simulink model "solar_pv_protected_c07_circuit"  (R2026b)
(part 4 of 16)

      | 用語9　　　　　　　 ; GND：Ground（回路の基準電位・電流帰路）。この図の共通基準。保護接地や大地への接続を意味するとは限らない。
      | 用語10　　　　　　　; AGND：Analog Ground（アナログ回路の基準端子）。アナログ部分の電流帰路。現図では共通GNDへ接続されるが、実装時の電流経路への配慮は別途必要。
      | 用語11　　　　　　　; DGND：Digital Ground（デジタル回路の基準端子）。デジタル部分の電流帰路。現図では共通GNDへ接続される。
      | 用語12　　　　　　　; VREF/REF：基準電圧を表す端子名。REFはReference（基準）の意味。ADCの変換尺度や電流アンプの出力基準に使う。REF1/REF2の接続電位は個別に確認する。
      | 用語13　　　　　　　; VCC/VDD/VEE/VS：ICの電源端子名。文字の歴史的な由来を現在の接続機能へ当てはめない。現回路のVEEはU8/U10では浮動基準SW、U9ではGND。各電圧・基準は端子と接続を参照する。
      | 用語14　　　　　　　; GNDP：U10の一次側電源の基準端子。絶縁電源の入力側GND。二次側基準VEE=SWと直接同一の導体ではない。
      | 用語15　　　　　　　; SW：Switching Node（スイッチング点）。主電力段の上下MOSFETとL1がつながる、電圧が高速に切り替わる点。GNDとは別電位。
  GND_Label_043 : ConnectionLabel  Description=|  Label=GND
      | この回路での名前　　; GND
      | 種別　　　　　　　　; ConnectionLabel
      | この回路での役割　　; 電池BT1の負極、太陽電池列の負極、制御・測定・保護回路のGNDを結ぶ共通の帰路。高側駆動の浮動帰路SWとは別のノード。
      | 共通帰路の代表接続　; BT1（充電先の蓄電池／51.2V 100Ah LiFePO4）: -
      |                     ; PV1（直列太陽電池列の負極側パネル／400W panel 1/2）: -
      |                     ; U7（RP2040搭載Pico W／SC0918）: 3(GND), 8(GND), 13(GND), 18(GND), 23(GND), 28(GND), 33(AGND), 38(GND)
      |                     ; U1（外付けADC／MCP3208-CI/SL）: 8(CH7), 9(DGND), 14(AGND)
      |                     ; P_U1（保護MOSFETを制御する保護IC／LTC4364IMS-1#PBF）: GND
      |                     ; Q2（同期整流降圧回路の下側スイッチ／TK9R6E15Q5,S1X）: 3(S)
      |                     ; U9（低側の光ゲートドライバ／ACPL-P346-560E）: 4(VEE)
      |                     ; U10（高側ゲート用の浮動電源を作る絶縁DC/DC／UCC14131QDWNRQ1）: 1(GNDP), 2(GNDP), 5(GNDP), 8(GNDP), 9(GNDP), 10(GNDP), 11(GNDP), 12(GNDP), 13(GNDP), 14(GNDP), 15(GNDP), 16(GNDP), 17(GNDP), 18(GNDP)
      | この場所の直接接続　; C7（入力フィルム／3.3 uF）: 2(n)
      | 直接接続の範囲　　　; このラベルから実際の線・分岐・明示的な境界端子だけを追った接続。同名ラベルによる離れた場所への接続はこの欄に含めない。
      | 同一ネット全端子　　; BT1: -
      |                     ; C1: 2(n)
      |                     ; C2: 2(n)
      |                     ; C3: 2(n)
      |                     ; C4: 2(n)
      |                     ; C7: 2(n)
      |                     ; C8: 2(n)
      |                     ; C9: 2(n)
      |                     ; C10: 2(n)
      |                     ; C13: 2(n)
      |                     ; C14: 2(n)
      |                     ; C15: 2(n)
      |                     ; C16: 2(n)
      |                     ; C17: 2
      |                     ; C18: 2
      |                     ; C19: 2
      |                     ; C20: 2
      |                     ; C21: 2
      |                     ; C22: 2
      |                     ; C23: 2
      |                     ; C24: 2
      |                     ; C25: 2
      |                     ; C26: 2
      |                     ; C27: 2
      |                     ; C28: 2
      |                     ; C29: 2
      |                     ; C30: 2
      |                     ; C31: 2
      |                     ; C33: 2
      |                     ; C34: 2
      |                     ; C35: 2
      |                     ; C36: 2
      |                     ; C40: 2
      |                     ; C41: 2
      |                     ; C42: 2
      |                     ; C43: 2
      |                     ; C44: 2
      |                     ; C45: 2
      |                     ; C46: 2
      |                     ; C47: 2
      |                     ; C48: 2
      |                     ; D2: 2(A)
      |                     ; PV1: -
      |                     ; P_CHG: N
      |                     ; P_COUT: N
      |                     ; P_CTMR: N
      |                     ; P_D1: A
      |                     ; P_R3: 2
      |                     ; P_R8: 2
      |                     ; P_RSHDN_PD: 2
      |                     ; P_U1: GND
      |                     ; Q2: 3(S)
      |                     ; Q3: 1(S1), 4(S2)
      |                     ; R1: 2(n)
      |                     ; R18: 2
      |                     ; R21: 2
      |                     ; R24: 2
      |                     ; R35: 2
      |                     ; R42: 2
      |                     ; R44: 2
      |                     ; R48: 2
      |                     ; U1: 8(CH7), 9(DGND), 14(AGND)
      |                     ; U2: 2(GND), 3(REF2), 4(RESERVED_GND)
      |                     ; U3: 2(GND), 3(REF2), 4(RESERVED_GND)
      |                     ; U4: 3(GND)
      |                     ; U5: 3(GND)
      |                     ; U6: 3(GND)
      |                     ; U7: 3(GND), 8(GND), 13(GND), 18(GND), 23(GND), 28(GND), 33(AGND), 38(GND)
      |                     ; U9: 4(VEE)
      |                     ; U10: 1(GNDP), 2(GNDP), 5(GNDP), 8(GNDP), 9(GNDP), 10(GNDP), 11(GNDP), 12(GNDP), 13(GNDP), 14(GNDP), 15(GNDP), 16(GNDP), 17(GNDP), 18(GNDP)
      |                     ; U11: 2(GND)
      |                     ; U12: 2(GND)
      | 接続部品数　　　　　; 72部品（部品番号で集計。同一ネット全体）
      | 接続端子数　　　　　; 99端子（423端子の部品対応表で集計。ラベル・境界ポートの重複は含めない）
      | この場所の端子数　　; 1端子／1部品（同名ラベルによる接続を除く）
      | 同階層同名ラベル数　; 75個（このラベル自身を含む）
      | 全階層の接続ラベル　; 87個（実際に同じノードへつながるラベル。名前が違う別名も含む）
      | 接続ルール　　　　　; 同じ階層の同じラベル名を仮想配線として結ぶ。別のSubsystem内とは名前だけでつながらず、明示的なConnection Portと配線をたどる。色は用途の表示であり接続を決めない。
      | 確認の範囲　　　　　; 現在の保存回路の端子・配線から求めた静的接続。抵抗やICの内部を導線として短絡せずに集計した。説明の更新は動作シミュレーション、タイミング、実部品の性能・実機動作を保証するものではない。
      | 記録の基準　　　　　; measurement_label_layout_20261022_r01/after_layout_graph.json。部品対応表は端子名の対応付けにのみ使用。
      | 
      | 【この説明欄の略語・記号】
      | 用語1　　　　　　　 ; DC：Direct Current（直流）。ここでは直流電源または直流成分。DCバイアスはコンデンサに重なる直流電圧を指す。
      | 用語2　　　　　　　 ; DC/DC：DC-to-DC Converter（直流電圧変換器）。直流入力を別の直流電圧へ変換する電源回路。絶縁の有無は個々の部品説明で確認する。
      | 用語3　　　　　　　 ; ADC：Analog-to-Digital Converter（アナログ・デジタル変換器）。測定電圧をデジタル値へ変換する回路。電流や温度も、センサーで電圧へ変換した後に読み取る。
      | 用語4　　　　　　　 ; IC：Integrated Circuit（集積回路）。複数の電子素子と機能を小さな半導体チップに集積した部品。
      | 用語5　　　　　　　 ; CH：Channel（測定チャネル）。CH0〜CH7はADCの入力番号であり、同時測定を意味しない。
      | 用語6　　　　　　　 ; MOSFET：Metal-Oxide-Semiconductor Field-Effect Transistor（金属・酸化膜・半導体構造の電界効果トランジスタ）。ゲートとソースの電圧でドレインとソースの導通を制御する素子。N-MOSはNチャネル型を表す。
      | 用語7　　　　　　　 ; LiFePO4：Lithium Iron Phosphate（リン酸鉄リチウム）。電池の正極材料を示す化学式。英語の頭文字を並べた略語ではない。
      | 用語8　　　　　　　 ; GND：Ground（回路の基準電位・電流帰路）。この図の共通基準。保護接地や大地への接続を意味するとは限らない。
      | 用語9　　　　　　　 ; AGND：Analog Ground（アナログ回路の基準端子）。アナログ部分の電流帰路。現図では共通GNDへ接続されるが、実装時の電流経路への配慮は別途必要。
      | 用語10　　　　　　　; DGND：Digital Ground（デジタル回路の基準端子）。デジタル部分の電流帰路。現図では共通GNDへ接続される。
      | 用語11　　　　　　　; VREF/REF：基準電圧を表す端子名。REFはReference（基準）の意味。ADCの変換尺度や電流アンプの出力基準に使う。REF1/REF2の接続電位は個別に確認する。
      | 用語12　　　　　　　; VCC/VDD/VEE/VS：ICの電源端子名。文字の歴史的な由来を現在の接続機能へ当てはめない。現回路のVEEはU8/U10では浮動基準SW、U9ではGND。各電圧・基準は端子と接続を参照する。
      | 用語13　　　　　　　; GNDP：U10の一次側電源の基準端子。絶縁電源の入力側GND。二次側基準VEE=SWと直接同一の導体ではない。
      | 用語14　　　　　　　; SW：Switching Node（スイッチング点）。主電力段の上下MOSFETとL1がつながる、電圧が高速に切り替わる点。GNDとは別電位。
  GND_Label_044 : ConnectionLabel  Description=|  Label=GND
      | この回路での名前　　; GND
      | 種別　　　　　　　　; ConnectionLabel
      | この回路での役割　　; 電池BT1の負極、太陽電池列の負極、制御・測定・保護回路のGNDを結ぶ共通の帰路。高側駆動の浮動帰路SWとは別のノード。
      | 共通帰路の代表接続　; BT1（充電先の蓄電池／51.2V 100Ah LiFePO4）: -
      |                     ; PV1（直列太陽電池列の負極側パネル／400W panel 1/2）: -
      |                     ; U7（RP2040搭載Pico W／SC0918）: 3(GND), 8(GND), 13(GND), 18(GND), 23(GND), 28(GND), 33(AGND), 38(GND)
      |                     ; U1（外付けADC／MCP3208-CI/SL）: 8(CH7), 9(DGND), 14(AGND)
      |                     ; P_U1（保護MOSFETを制御する保護IC／LTC4364IMS-1#PBF）: GND
      |                     ; Q2（同期整流降圧回路の下側スイッチ／TK9R6E15Q5,S1X）: 3(S)
      |                     ; U9（低側の光ゲートドライバ／ACPL-P346-560E）: 4(VEE)
      |                     ; U10（高側ゲート用の浮動電源を作る絶縁DC/DC／UCC14131QDWNRQ1）: 1(GNDP), 2(GNDP), 5(GNDP), 8(GNDP), 9(GNDP), 10(GNDP), 11(GNDP), 12(GNDP), 13(GNDP), 14(GNDP), 15(GNDP), 16(GNDP), 17(GNDP), 18(GNDP)
      | この場所の直接接続　; C8（入力高速バイパス／2.2 uF）: 2(n)
      | 直接接続の範囲　　　; このラベルから実際の線・分岐・明示的な境界端子だけを追った接続。同名ラベルによる離れた場所への接続はこの欄に含めない。
      | 同一ネット全端子　　; BT1: -
      |                     ; C1: 2(n)
      |                     ; C2: 2(n)
      |                     ; C3: 2(n)
      |                     ; C4: 2(n)
      |                     ; C7: 2(n)
      |                     ; C8: 2(n)
      |                     ; C9: 2(n)
      |                     ; C10: 2(n)
      |                     ; C13: 2(n)
      |                     ; C14: 2(n)
      |                     ; C15: 2(n)
      |                     ; C16: 2(n)
      |                     ; C17: 2
      |                     ; C18: 2
      |                     ; C19: 2
      |                     ; C20: 2
      |                     ; C21: 2
      |                     ; C22: 2
      |                     ; C23: 2
      |                     ; C24: 2
      |                     ; C25: 2
      |                     ; C26: 2
      |                     ; C27: 2
      |                     ; C28: 2
      |                     ; C29: 2
      |                     ; C30: 2
      |                     ; C31: 2
      |                     ; C33: 2
      |                     ; C34: 2
      |                     ; C35: 2
      |                     ; C36: 2
      |                     ; C40: 2
      |                     ; C41: 2
      |                     ; C42: 2
      |                     ; C43: 2
      |                     ; C44: 2
      |                     ; C45: 2
      |                     ; C46: 2
      |                     ; C47: 2
      |                     ; C48: 2
      |                     ; D2: 2(A)
      |                     ; PV1: -
      |                     ; P_CHG: N
      |                     ; P_COUT: N
      |                     ; P_CTMR: N
      |                     ; P_D1: A
      |                     ; P_R3: 2
      |                     ; P_R8: 2
      |                     ; P_RSHDN_PD: 2
      |                     ; P_U1: GND
      |                     ; Q2: 3(S)
      |                     ; Q3: 1(S1), 4(S2)
      |                     ; R1: 2(n)
      |                     ; R18: 2
      |                     ; R21: 2
      |                     ; R24: 2
      |                     ; R35: 2
      |                     ; R42: 2
      |                     ; R44: 2
      |                     ; R48: 2
      |                     ; U1: 8(CH7), 9(DGND), 14(AGND)
      |                     ; U2: 2(GND), 3(REF2), 4(RESERVED_GND)
      |                     ; U3: 2(GND), 3(REF2), 4(RESERVED_GND)
      |                     ; U4: 3(GND)
      |                     ; U5: 3(GND)
      |                     ; U6: 3(GND)
      |                     ; U7: 3(GND), 8(GND), 13(GND), 18(GND), 23(GND), 28(GND), 33(AGND), 38(GND)
      |                     ; U9: 4(VEE)
      |                     ; U10: 1(GNDP), 2(GNDP), 5(GNDP), 8(GNDP), 9(GNDP), 10(GNDP), 11(GNDP), 12(GNDP), 13(GNDP), 14(GNDP), 15(GNDP), 16(GNDP), 17(GNDP), 18(GNDP)
      |                     ; U11: 2(GND)
      |                     ; U12: 2(GND)
      | 接続部品数　　　　　; 72部品（部品番号で集計。同一ネット全体）
      | 接続端子数　　　　　; 99端子（423端子の部品対応表で集計。ラベル・境界ポートの重複は含めない）
      | この場所の端子数　　; 1端子／1部品（同名ラベルによる接続を除く）
      | 同階層同名ラベル数　; 75個（このラベル自身を含む）
      | 全階層の接続ラベル　; 87個（実際に同じノードへつながるラベル。名前が違う別名も含む）
      | 接続ルール　　　　　; 同じ階層の同じラベル名を仮想配線として結ぶ。別のSubsystem内とは名前だけでつながらず、明示的なConnection Portと配線をたどる。色は用途の表示であり接続を決めない。
      | 確認の範囲　　　　　; 現在の保存回路の端子・配線から求めた静的接続。抵抗やICの内部を導線として短絡せずに集計した。説明の更新は動作シミュレーション、タイミング、実部品の性能・実機動作を保証するものではない。
      | 記録の基準　　　　　; measurement_label_layout_20261022_r01/after_layout_graph.json。部品対応表は端子名の対応付けにのみ使用。
      | 
      | 【この説明欄の略語・記号】
      | 用語1　　　　　　　 ; DC：Direct Current（直流）。ここでは直流電源または直流成分。DCバイアスはコンデンサに重なる直流電圧を指す。
      | 用語2　　　　　　　 ; DC/DC：DC-to-DC Converter（直流電圧変換器）。直流入力を別の直流電圧へ変換する電源回路。絶縁の有無は個々の部品説明で確認する。
      | 用語3　　　　　　　 ; ADC：Analog-to-Digital Converter（アナログ・デジタル変換器）。測定電圧をデジタル値へ変換する回路。電流や温度も、センサーで電圧へ変換した後に読み取る。
      | 用語4　　　　　　　 ; IC：Integrated Circuit（集積回路）。複数の電子素子と機能を小さな半導体チップに集積した部品。
      | 用語5　　　　　　　 ; CH：Channel（測定チャネル）。CH0〜CH7はADCの入力番号であり、同時測定を意味しない。
      | 用語6　　　　　　　 ; MOSFET：Metal-Oxide-Semiconductor Field-Effect Transistor（金属・酸化膜・半導体構造の電界効果トランジスタ）。ゲートとソースの電圧でドレインとソースの導通を制御する素子。N-MOSはNチャネル型を表す。
      | 用語7　　　　　　　 ; LiFePO4：Lithium Iron Phosphate（リン酸鉄リチウム）。電池の正極材料を示す化学式。英語の頭文字を並べた略語ではない。
      | 用語8　　　　　　　 ; GND：Ground（回路の基準電位・電流帰路）。この図の共通基準。保護接地や大地への接続を意味するとは限らない。
      | 用語9　　　　　　　 ; AGND：Analog Ground（アナログ回路の基準端子）。アナログ部分の電流帰路。現図では共通GNDへ接続されるが、実装時の電流経路への配慮は別途必要。
      | 用語10　　　　　　　; DGND：Digital Ground（デジタル回路の基準端子）。デジタル部分の電流帰路。現図では共通GNDへ接続される。
      | 用語11　　　　　　　; VREF/REF：基準電圧を表す端子名。REFはReference（基準）の意味。ADCの変換尺度や電流アンプの出力基準に使う。REF1/REF2の接続電位は個別に確認する。
      | 用語12　　　　　　　; VCC/VDD/VEE/VS：ICの電源端子名。文字の歴史的な由来を現在の接続機能へ当てはめない。現回路のVEEはU8/U10では浮動基準SW、U9ではGND。各電圧・基準は端子と接続を参照する。
      | 用語13　　　　　　　; GNDP：U10の一次側電源の基準端子。絶縁電源の入力側GND。二次側基準VEE=SWと直接同一の導体ではない。
      | 用語14　　　　　　　; SW：Switching Node（スイッチング点）。主電力段の上下MOSFETとL1がつながる、電圧が高速に切り替わる点。GNDとは別電位。
  GND_Label_045 : ConnectionLabel  Description=|  Label=GND
      | この回路での名前　　; GND
      | 種別　　　　　　　　; ConnectionLabel
      | この回路での役割　　; 電池BT1の負極、太陽電池列の負極、制御・測定・保護回路のGNDを結ぶ共通の帰路。高側駆動の浮動帰路SWとは別のノード。
      | 共通帰路の代表接続　; BT1（充電先の蓄電池／51.2V 100Ah LiFePO4）: -
      |                     ; PV1（直列太陽電池列の負極側パネル／400W panel 1/2）: -
      |                     ; U7（RP2040搭載Pico W／SC0918）: 3(GND), 8(GND), 13(GND), 18(GND), 23(GND), 28(GND), 33(AGND), 38(GND)
      |                     ; U1（外付けADC／MCP3208-CI/SL）: 8(CH7), 9(DGND), 14(AGND)
      |                     ; P_U1（保護MOSFETを制御する保護IC／LTC4364IMS-1#PBF）: GND
      |                     ; Q2（同期整流降圧回路の下側スイッチ／TK9R6E15Q5,S1X）: 3(S)
      |                     ; U9（低側の光ゲートドライバ／ACPL-P346-560E）: 4(VEE)
      |                     ; U10（高側ゲート用の浮動電源を作る絶縁DC/DC／UCC14131QDWNRQ1）: 1(GNDP), 2(GNDP), 5(GNDP), 8(GNDP), 9(GNDP), 10(GNDP), 11(GNDP), 12(GNDP), 13(GNDP), 14(GNDP), 15(GNDP), 16(GNDP), 17(GNDP), 18(GNDP)
      | この場所の直接接続　; C9（入力高速バイパス／2.2 uF）: 2(n)
      | 直接接続の範囲　　　; このラベルから実際の線・分岐・明示的な境界端子だけを追った接続。同名ラベルによる離れた場所への接続はこの欄に含めない。
      | 同一ネット全端子　　; BT1: -
      |                     ; C1: 2(n)
      |                     ; C2: 2(n)
      |                     ; C3: 2(n)
      |                     ; C4: 2(n)
      |                     ; C7: 2(n)
      |                     ; C8: 2(n)
      |                     ; C9: 2(n)
      |                     ; C10: 2(n)
      |                     ; C13: 2(n)
      |                     ; C14: 2(n)
      |                     ; C15: 2(n)
      |                     ; C16: 2(n)
      |                     ; C17: 2
      |                     ; C18: 2
      |                     ; C19: 2
      |                     ; C20: 2
      |                     ; C21: 2
      |                     ; C22: 2
      |                     ; C23: 2
      |                     ; C24: 2
      |                     ; C25: 2
      |                     ; C26: 2
      |                     ; C27: 2
      |                     ; C28: 2
      |                     ; C29: 2
      |                     ; C30: 2
      |                     ; C31: 2
      |                     ; C33: 2
      |                     ; C34: 2
      |                     ; C35: 2
      |                     ; C36: 2
      |                     ; C40: 2
      |                     ; C41: 2
      |                     ; C42: 2
      |                     ; C43: 2
      |                     ; C44: 2
      |                     ; C45: 2
      |                     ; C46: 2
      |                     ; C47: 2
      |                     ; C48: 2
      |                     ; D2: 2(A)
      |                     ; PV1: -
      |                     ; P_CHG: N
      |                     ; P_COUT: N
      |                     ; P_CTMR: N
      |                     ; P_D1: A
      |                     ; P_R3: 2
      |                     ; P_R8: 2
      |                     ; P_RSHDN_PD: 2
      |                     ; P_U1: GND
      |                     ; Q2: 3(S)
      |                     ; Q3: 1(S1), 4(S2)
      |                     ; R1: 2(n)
      |                     ; R18: 2
      |                     ; R21: 2
      |                     ; R24: 2
      |                     ; R35: 2
      |                     ; R42: 2
      |                     ; R44: 2
      |                     ; R48: 2
      |                     ; U1: 8(CH7), 9(DGND), 14(AGND)
      |                     ; U2: 2(GND), 3(REF2), 4(RESERVED_GND)
      |                     ; U3: 2(GND), 3(REF2), 4(RESERVED_GND)
      |                     ; U4: 3(GND)
      |                     ; U5: 3(GND)
      |                     ; U6: 3(GND)
      |                     ; U7: 3(GND), 8(GND), 13(GND), 18(GND), 23(GND), 28(GND), 33(AGND), 38(GND)
      |                     ; U9: 4(VEE)
      |                     ; U10: 1(GNDP), 2(GNDP), 5(GNDP), 8(GNDP), 9(GNDP), 10(GNDP), 11(GNDP), 12(GNDP), 13(GNDP), 14(GNDP), 15(GNDP), 16(GNDP), 17(GNDP), 18(GNDP)
      |                     ; U11: 2(GND)
      |                     ; U12: 2(GND)
      | 接続部品数　　　　　; 72部品（部品番号で集計。同一ネット全体）
      | 接続端子数　　　　　; 99端子（423端子の部品対応表で集計。ラベル・境界ポートの重複は含めない）
      | この場所の端子数　　; 1端子／1部品（同名ラベルによる接続を除く）
      | 同階層同名ラベル数　; 75個（このラベル自身を含む）
      | 全階層の接続ラベル　; 87個（実際に同じノードへつながるラベル。名前が違う別名も含む）
      | 接続ルール　　　　　; 同じ階層の同じラベル名を仮想配線として結ぶ。別のSubsystem内とは名前だけでつながらず、明示的なConnection Portと配線をたどる。色は用途の表示であり接続を決めない。
      | 確認の範囲　　　　　; 現在の保存回路の端子・配線から求めた静的接続。抵抗やICの内部を導線として短絡せずに集計した。説明の更新は動作シミュレーション、タイミング、実部品の性能・実機動作を保証するものではない。
      | 記録の基準　　　　　; measurement_label_layout_20261022_r01/after_layout_graph.json。部品対応表は端子名の対応付けにのみ使用。
      | 
      | 【この説明欄の略語・記号】
      | 用語1　　　　　　　 ; DC：Direct Current（直流）。ここでは直流電源または直流成分。DCバイアスはコンデンサに重なる直流電圧を指す。
      | 用語2　　　　　　　 ; DC/DC：DC-to-DC Converter（直流電圧変換器）。直流入力を別の直流電圧へ変換する電源回路。絶縁の有無は個々の部品説明で確認する。
      | 用語3　　　　　　　 ; ADC：Analog-to-Digital Converter（アナログ・デジタル変換器）。測定電圧をデジタル値へ変換する回路。電流や温度も、センサーで電圧へ変換した後に読み取る。
      | 用語4　　　　　　　 ; IC：Integrated Circuit（集積回路）。複数の電子素子と機能を小さな半導体チップに集積した部品。
      | 用語5　　　　　　　 ; CH：Channel（測定チャネル）。CH0〜CH7はADCの入力番号であり、同時測定を意味しない。
      | 用語6　　　　　　　 ; MOSFET：Metal-Oxide-Semiconductor Field-Effect Transistor（金属・酸化膜・半導体構造の電界効果トランジスタ）。ゲートとソースの電圧でドレインとソースの導通を制御する素子。N-MOSはNチャネル型を表す。
      | 用語7　　　　　　　 ; LiFePO4：Lithium Iron Phosphate（リン酸鉄リチウム）。電池の正極材料を示す化学式。英語の頭文字を並べた略語ではない。
      | 用語8　　　　　　　 ; GND：Ground（回路の基準電位・電流帰路）。この図の共通基準。保護接地や大地への接続を意味するとは限らない。
      | 用語9　　　　　　　 ; AGND：Analog Ground（アナログ回路の基準端子）。アナログ部分の電流帰路。現図では共通GNDへ接続されるが、実装時の電流経路への配慮は別途必要。
      | 用語10　　　　　　　; DGND：Digital Ground（デジタル回路の基準端子）。デジタル部分の電流帰路。現図では共通GNDへ接続される。
      | 用語11　　　　　　　; VREF/REF：基準電圧を表す端子名。REFはReference（基準）の意味。ADCの変換尺度や電流アンプの出力基準に使う。REF1/REF2の接続電位は個別に確認する。
      | 用語12　　　　　　　; VCC/VDD/VEE/VS：ICの電源端子名。文字の歴史的な由来を現在の接続機能へ当てはめない。現回路のVEEはU8/U10では浮動基準SW、U9ではGND。各電圧・基準は端子と接続を参照する。
      | 用語13　　　　　　　; GNDP：U10の一次側電源の基準端子。絶縁電源の入力側GND。二次側基準VEE=SWと直接同一の導体ではない。
      | 用語14　　　　　　　; SW：Switching Node（スイッチング点）。主電力段の上下MOSFETとL1がつながる、電圧が高速に切り替わる点。GNDとは別電位。
  GND_Label_046 : ConnectionLabel  Description=|  Label=GND
      | この回路での名前　　; GND
      | 種別　　　　　　　　; ConnectionLabel
      | この回路での役割　　; 電池BT1の負極、太陽電池列の負極、制御・測定・保護回路のGNDを結ぶ共通の帰路。高側駆動の浮動帰路SWとは別のノード。
      | 共通帰路の代表接続　; BT1（充電先の蓄電池／51.2V 100Ah LiFePO4）: -
      |                     ; PV1（直列太陽電池列の負極側パネル／400W panel 1/2）: -
      |                     ; U7（RP2040搭載Pico W／SC0918）: 3(GND), 8(GND), 13(GND), 18(GND), 23(GND), 28(GND), 33(AGND), 38(GND)
      |                     ; U1（外付けADC／MCP3208-CI/SL）: 8(CH7), 9(DGND), 14(AGND)
      |                     ; P_U1（保護MOSFETを制御する保護IC／LTC4364IMS-1#PBF）: GND
      |                     ; Q2（同期整流降圧回路の下側スイッチ／TK9R6E15Q5,S1X）: 3(S)
      |                     ; U9（低側の光ゲートドライバ／ACPL-P346-560E）: 4(VEE)
      |                     ; U10（高側ゲート用の浮動電源を作る絶縁DC/DC／UCC14131QDWNRQ1）: 1(GNDP), 2(GNDP), 5(GNDP), 8(GNDP), 9(GNDP), 10(GNDP), 11(GNDP), 12(GNDP), 13(GNDP), 14(GNDP), 15(GNDP), 16(GNDP), 17(GNDP), 18(GNDP)
      | この場所の直接接続　; D2（Q2のゲート–ソース間電圧が過大になるのを抑えるため、GATE_L–GND間へ配置する／15V gate clamp）: 2(A)
      |                     ; Q2（同期整流降圧回路の下側スイッチ／TK9R6E15Q5,S1X）: 3(S)
      |                     ; R44（Q2のゲートをソースGNDへ戻し、ドライバ未給電時の残留電荷を逃がす／10k 1%）: 2
      | 直接接続の範囲　　　; このラベルから実際の線・分岐・明示的な境界端子だけを追った接続。同名ラベルによる離れた場所への接続はこの欄に含めない。
      | 同一ネット全端子　　; BT1: -
      |                     ; C1: 2(n)
      |                     ; C2: 2(n)
      |                     ; C3: 2(n)
      |                     ; C4: 2(n)
      |                     ; C7: 2(n)
      |                     ; C8: 2(n)
      |                     ; C9: 2(n)
      |                     ; C10: 2(n)
      |                     ; C13: 2(n)
      |                     ; C14: 2(n)
      |                     ; C15: 2(n)
      |                     ; C16: 2(n)
      |                     ; C17: 2
      |                     ; C18: 2
      |                     ; C19: 2
      |                     ; C20: 2
      |                     ; C21: 2
      |                     ; C22: 2
      |                     ; C23: 2
      |                     ; C24: 2
      |                     ; C25: 2
      |                     ; C26: 2
      |                     ; C27: 2
      |                     ; C28: 2
      |                     ; C29: 2
      |                     ; C30: 2
      |                     ; C31: 2
      |                     ; C33: 2
      |                     ; C34: 2
      |                     ; C35: 2
      |                     ; C36: 2
      |                     ; C40: 2
      |                     ; C41: 2
      |                     ; C42: 2
      |                     ; C43: 2
      |                     ; C44: 2
      |                     ; C45: 2
      |                     ; C46: 2
      |                     ; C47: 2
      |                     ; C48: 2
      |                     ; D2: 2(A)
      |                     ; PV1: -
      |                     ; P_CHG: N
      |                     ; P_COUT: N
      |                     ; P_CTMR: N
      |                     ; P_D1: A
      |                     ; P_R3: 2
      |                     ; P_R8: 2
      |                     ; P_RSHDN_PD: 2
      |                     ; P_U1: GND
      |                     ; Q2: 3(S)
      |                     ; Q3: 1(S1), 4(S2)
      |                     ; R1: 2(n)
      |                     ; R18: 2
      |                     ; R21: 2
      |                     ; R24: 2
      |                     ; R35: 2
      |                     ; R42: 2
      |                     ; R44: 2
      |                     ; R48: 2
      |                     ; U1: 8(CH7), 9(DGND), 14(AGND)
      |                     ; U2: 2(GND), 3(REF2), 4(RESERVED_GND)
      |                     ; U3: 2(GND), 3(REF2), 4(RESERVED_GND)
      |                     ; U4: 3(GND)
      |                     ; U5: 3(GND)
      |                     ; U6: 3(GND)
      |                     ; U7: 3(GND), 8(GND), 13(GND), 18(GND), 23(GND), 28(GND), 33(AGND), 38(GND)
      |                     ; U9: 4(VEE)
      |                     ; U10: 1(GNDP), 2(GNDP), 5(GNDP), 8(GNDP), 9(GNDP), 10(GNDP), 11(GNDP), 12(GNDP), 13(GNDP), 14(GNDP), 15(GNDP), 16(GNDP), 17(GNDP), 18(GNDP)
      |                     ; U11: 2(GND)
      |                     ; U12: 2(GND)
      | 接続部品数　　　　　; 72部品（部品番号で集計。同一ネット全体）
      | 接続端子数　　　　　; 99端子（423端子の部品対応表で集計。ラベル・境界ポートの重複は含めない）
      | この場所の端子数　　; 3端子／3部品（同名ラベルによる接続を除く）
      | 同階層同名ラベル数　; 75個（このラベル自身を含む）
      | 全階層の接続ラベル　; 87個（実際に同じノードへつながるラベル。名前が違う別名も含む）
      | 接続ルール　　　　　; 同じ階層の同じラベル名を仮想配線として結ぶ。別のSubsystem内とは名前だけでつながらず、明示的なConnection Portと配線をたどる。色は用途の表示であり接続を決めない。
      | 確認の範囲　　　　　; 現在の保存回路の端子・配線から求めた静的接続。抵抗やICの内部を導線として短絡せずに集計した。説明の更新は動作シミュレーション、タイミング、実部品の性能・実機動作を保証するものではない。
      | 記録の基準　　　　　; measurement_label_layout_20261022_r01/after_layout_graph.json。部品対応表は端子名の対応付けにのみ使用。
      | 
      | 【この説明欄の略語・記号】
      | 用語1　　　　　　　 ; DC：Direct Current（直流）。ここでは直流電源または直流成分。DCバイアスはコンデンサに重なる直流電圧を指す。
      | 用語2　　　　　　　 ; DC/DC：DC-to-DC Converter（直流電圧変換器）。直流入力を別の直流電圧へ変換する電源回路。絶縁の有無は個々の部品説明で確認する。
      | 用語3　　　　　　　 ; ADC：Analog-to-Digital Converter（アナログ・デジタル変換器）。測定電圧をデジタル値へ変換する回路。電流や温度も、センサーで電圧へ変換した後に読み取る。
      | 用語4　　　　　　　 ; IC：Integrated Circuit（集積回路）。複数の電子素子と機能を小さな半導体チップに集積した部品。
      | 用語5　　　　　　　 ; CH：Channel（測定チャネル）。CH0〜CH7はADCの入力番号であり、同時測定を意味しない。
      | 用語6　　　　　　　 ; MOSFET：Metal-Oxide-Semiconductor Field-Effect Transistor（金属・酸化膜・半導体構造の電界効果トランジスタ）。ゲートとソースの電圧でドレインとソースの導通を制御する素子。N-MOSはNチャネル型を表す。
      | 用語7　　　　　　　 ; LiFePO4：Lithium Iron Phosphate（リン酸鉄リチウム）。電池の正極材料を示す化学式。英語の頭文字を並べた略語ではない。
      | 用語8　　　　　　　 ; GND：Ground（回路の基準電位・電流帰路）。この図の共通基準。保護接地や大地への接続を意味するとは限らない。
      | 用語9　　　　　　　 ; AGND：Analog Ground（アナログ回路の基準端子）。アナログ部分の電流帰路。現図では共通GNDへ接続されるが、実装時の電流経路への配慮は別途必要。
      | 用語10　　　　　　　; DGND：Digital Ground（デジタル回路の基準端子）。デジタル部分の電流帰路。現図では共通GNDへ接続される。
      | 用語11　　　　　　　; VREF/REF：基準電圧を表す端子名。REFはReference（基準）の意味。ADCの変換尺度や電流アンプの出力基準に使う。REF1/REF2の接続電位は個別に確認する。
      | 用語12　　　　　　　; VCC/VDD/VEE/VS：ICの電源端子名。文字の歴史的な由来を現在の接続機能へ当てはめない。現回路のVEEはU8/U10では浮動基準SW、U9ではGND。各電圧・基準は端子と接続を参照する。
      | 用語13　　　　　　　; GNDP：U10の一次側電源の基準端子。絶縁電源の入力側GND。二次側基準VEE=SWと直接同一の導体ではない。
      | 用語14　　　　　　　; SW：Switching Node（スイッチング点）。主電力段の上下MOSFETとL1がつながる、電圧が高速に切り替わる点。GNDとは別電位。
  GND_Label_047 : ConnectionLabel  Description=|  Label=GND
      | この回路での名前　　; GND
      | 種別　　　　　　　　; ConnectionLabel
      | この回路での役割　　; 電池BT1の負極、太陽電池列の負極、制御・測定・保護回路のGNDを結ぶ共通の帰路。高側駆動の浮動帰路SWとは別のノード。
      | 共通帰路の代表接続　; BT1（充電先の蓄電池／51.2V 100Ah LiFePO4）: -
      |                     ; PV1（直列太陽電池列の負極側パネル／400W panel 1/2）: -
      |                     ; U7（RP2040搭載Pico W／SC0918）: 3(GND), 8(GND), 13(GND), 18(GND), 23(GND), 28(GND), 33(AGND), 38(GND)
      |                     ; U1（外付けADC／MCP3208-CI/SL）: 8(CH7), 9(DGND), 14(AGND)
      |                     ; P_U1（保護MOSFETを制御する保護IC／LTC4364IMS-1#PBF）: GND
      |                     ; Q2（同期整流降圧回路の下側スイッチ／TK9R6E15Q5,S1X）: 3(S)
      |                     ; U9（低側の光ゲートドライバ／ACPL-P346-560E）: 4(VEE)
      |                     ; U10（高側ゲート用の浮動電源を作る絶縁DC/DC／UCC14131QDWNRQ1）: 1(GNDP), 2(GNDP), 5(GNDP), 8(GNDP), 9(GNDP), 10(GNDP), 11(GNDP), 12(GNDP), 13(GNDP), 14(GNDP), 15(GNDP), 16(GNDP), 17(GNDP), 18(GNDP)
      | この場所の直接接続　; PV1（直列太陽電池列の負極側パネル／400W panel 1/2）: -
      | 直接接続の範囲　　　; このラベルから実際の線・分岐・明示的な境界端子だけを追った接続。同名ラベルによる離れた場所への接続はこの欄に含めない。
      | 同一ネット全端子　　; BT1: -
      |                     ; C1: 2(n)
      |                     ; C2: 2(n)
      |                     ; C3: 2(n)
      |                     ; C4: 2(n)
      |                     ; C7: 2(n)
      |                     ; C8: 2(n)
      |                     ; C9: 2(n)
      |                     ; C10: 2(n)
      |                     ; C13: 2(n)
      |                     ; C14: 2(n)
      |                     ; C15: 2(n)
      |                     ; C16: 2(n)
      |                     ; C17: 2
      |                     ; C18: 2
      |                     ; C19: 2
      |                     ; C20: 2
      |                     ; C21: 2
      |                     ; C22: 2
      |                     ; C23: 2
      |                     ; C24: 2
      |                     ; C25: 2
      |                     ; C26: 2
      |                     ; C27: 2
      |                     ; C28: 2
      |                     ; C29: 2
      |                     ; C30: 2
      |                     ; C31: 2
      |                     ; C33: 2
      |                     ; C34: 2
      |                     ; C35: 2
      |                     ; C36: 2
      |                     ; C40: 2
      |                     ; C41: 2
      |                     ; C42: 2
      |                     ; C43: 2
      |                     ; C44: 2
      |                     ; C45: 2
      |                     ; C46: 2
      |                     ; C47: 2
      |                     ; C48: 2
      |                     ; D2: 2(A)
      |                     ; PV1: -
      |                     ; P_CHG: N
      |                     ; P_COUT: N
      |                     ; P_CTMR: N
      |                     ; P_D1: A
      |                     ; P_R3: 2
      |                     ; P_R8: 2
      |                     ; P_RSHDN_PD: 2
      |                     ; P_U1: GND
      |                     ; Q2: 3(S)
      |                     ; Q3: 1(S1), 4(S2)
      |                     ; R1: 2(n)
      |                     ; R18: 2
      |                     ; R21: 2
      |                     ; R24: 2
      |                     ; R35: 2
      |                     ; R42: 2
      |                     ; R44: 2
      |                     ; R48: 2
      |                     ; U1: 8(CH7), 9(DGND), 14(AGND)
      |                     ; U2: 2(GND), 3(REF2), 4(RESERVED_GND)
      |                     ; U3: 2(GND), 3(REF2), 4(RESERVED_GND)
      |                     ; U4: 3(GND)
      |                     ; U5: 3(GND)
      |                     ; U6: 3(GND)
      |                     ; U7: 3(GND), 8(GND), 13(GND), 18(GND), 23(GND), 28(GND), 33(AGND), 38(GND)
      |                     ; U9: 4(VEE)
      |                     ; U10: 1(GNDP), 2(GNDP), 5(GNDP), 8(GNDP), 9(GNDP), 10(GNDP), 11(GNDP), 12(GNDP), 13(GNDP), 14(GNDP), 15(GNDP), 16(GNDP), 17(GNDP), 18(GNDP)
      |                     ; U11: 2(GND)
      |                     ; U12: 2(GND)
      | 接続部品数　　　　　; 72部品（部品番号で集計。同一ネット全体）
      | 接続端子数　　　　　; 99端子（423端子の部品対応表で集計。ラベル・境界ポートの重複は含めない）
      | この場所の端子数　　; 1端子／1部品（同名ラベルによる接続を除く）
      | 同階層同名ラベル数　; 75個（このラベル自身を含む）
      | 全階層の接続ラベル　; 87個（実際に同じノードへつながるラベル。名前が違う別名も含む）
      | 接続ルール　　　　　; 同じ階層の同じラベル名を仮想配線として結ぶ。別のSubsystem内とは名前だけでつながらず、明示的なConnection Portと配線をたどる。色は用途の表示であり接続を決めない。
      | 確認の範囲　　　　　; 現在の保存回路の端子・配線から求めた静的接続。抵抗やICの内部を導線として短絡せずに集計した。説明の更新は動作シミュレーション、タイミング、実部品の性能・実機動作を保証するものではない。
      | 記録の基準　　　　　; measurement_label_layout_20261022_r01/after_layout_graph.json。部品対応表は端子名の対応付けにのみ使用。
      | 
      | 【この説明欄の略語・記号】
      | 用語1　　　　　　　 ; DC：Direct Current（直流）。ここでは直流電源または直流成分。DCバイアスはコンデンサに重なる直流電圧を指す。
      | 用語2　　　　　　　 ; DC/DC：DC-to-DC Converter（直流電圧変換器）。直流入力を別の直流電圧へ変換する電源回路。絶縁の有無は個々の部品説明で確認する。
      | 用語3　　　　　　　 ; ADC：Analog-to-Digital Converter（アナログ・デジタル変換器）。測定電圧をデジタル値へ変換する回路。電流や温度も、センサーで電圧へ変換した後に読み取る。
      | 用語4　　　　　　　 ; IC：Integrated Circuit（集積回路）。複数の電子素子と機能を小さな半導体チップに集積した部品。
      | 用語5　　　　　　　 ; CH：Channel（測定チャネル）。CH0〜CH7はADCの入力番号であり、同時測定を意味しない。
      | 用語6　　　　　　　 ; MOSFET：Metal-Oxide-Semiconductor Field-Effect Transistor（金属・酸化膜・半導体構造の電界効果トランジスタ）。ゲートとソースの電圧でドレインとソースの導通を制御する素子。N-MOSはNチャネル型を表す。
      | 用語7　　　　　　　 ; LiFePO4：Lithium Iron Phosphate（リン酸鉄リチウム）。電池の正極材料を示す化学式。英語の頭文字を並べた略語ではない。
      | 用語8　　　　　　　 ; GND：Ground（回路の基準電位・電流帰路）。この図の共通基準。保護接地や大地への接続を意味するとは限らない。
      | 用語9　　　　　　　 ; AGND：Analog Ground（アナログ回路の基準端子）。アナログ部分の電流帰路。現図では共通GNDへ接続されるが、実装時の電流経路への配慮は別途必要。
      | 用語10　　　　　　　; DGND：Digital Ground（デジタル回路の基準端子）。デジタル部分の電流帰路。現図では共通GNDへ接続される。
      | 用語11　　　　　　　; VREF/REF：基準電圧を表す端子名。REFはReference（基準）の意味。ADCの変換尺度や電流アンプの出力基準に使う。REF1/REF2の接続電位は個別に確認する。
      | 用語12　　　　　　　; VCC/VDD/VEE/VS：ICの電源端子名。文字の歴史的な由来を現在の接続機能へ当てはめない。現回路のVEEはU8/U10では浮動基準SW、U9ではGND。各電圧・基準は端子と接続を参照する。
      | 用語13　　　　　　　; GNDP：U10の一次側電源の基準端子。絶縁電源の入力側GND。二次側基準VEE=SWと直接同一の導体ではない。
      | 用語14　　　　　　　; SW：Switching Node（スイッチング点）。主電力段の上下MOSFETとL1がつながる、電圧が高速に切り替わる点。GNDとは別電位。
  GND_Label_049 : ConnectionLabel  Description=|  Label=GND
      | この回路での名前　　; GND
      | 種別　　　　　　　　; ConnectionLabel
      | この回路での役割　　; 電池BT1の負極、太陽電池列の負極、制御・測定・保護回路のGNDを結ぶ共通の帰路。高側駆動の浮動帰路SWとは別のノード。
      | 共通帰路の代表接続　; BT1（充電先の蓄電池／51.2V 100Ah LiFePO4）: -
      |                     ; PV1（直列太陽電池列の負極側パネル／400W panel 1/2）: -
      |                     ; U7（RP2040搭載Pico W／SC0918）: 3(GND), 8(GND), 13(GND), 18(GND), 23(GND), 28(GND), 33(AGND), 38(GND)
      |                     ; U1（外付けADC／MCP3208-CI/SL）: 8(CH7), 9(DGND), 14(AGND)
      |                     ; P_U1（保護MOSFETを制御する保護IC／LTC4364IMS-1#PBF）: GND
      |                     ; Q2（同期整流降圧回路の下側スイッチ／TK9R6E15Q5,S1X）: 3(S)
      |                     ; U9（低側の光ゲートドライバ／ACPL-P346-560E）: 4(VEE)
      |                     ; U10（高側ゲート用の浮動電源を作る絶縁DC/DC／UCC14131QDWNRQ1）: 1(GNDP), 2(GNDP), 5(GNDP), 8(GNDP), 9(GNDP), 10(GNDP), 11(GNDP), 12(GNDP), 13(GNDP), 14(GNDP), 15(GNDP), 16(GNDP), 17(GNDP), 18(GNDP)
      | この場所の直接接続　; Q3（RP2040のPWM_Lを受け、U9の入力LED電流をGNDへ引き込む／dual 30V logic-level LED sink）: 1(S1)
      | 直接接続の範囲　　　; このラベルから実際の線・分岐・明示的な境界端子だけを追った接続。同名ラベルによる離れた場所への接続はこの欄に含めない。
      | 同一ネット全端子　　; BT1: -
      |                     ; C1: 2(n)
      |                     ; C2: 2(n)
      |                     ; C3: 2(n)
      |                     ; C4: 2(n)
      |                     ; C7: 2(n)
      |                     ; C8: 2(n)
      |                     ; C9: 2(n)
      |                     ; C10: 2(n)
      |                     ; C13: 2(n)
      |                     ; C14: 2(n)
      |                     ; C15: 2(n)
      |                     ; C16: 2(n)
      |                     ; C17: 2
      |                     ; C18: 2
      |                     ; C19: 2
      |                     ; C20: 2
      |                     ; C21: 2
      |                     ; C22: 2
      |                     ; C23: 2
      |                     ; C24: 2
      |                     ; C25: 2
      |                     ; C26: 2
      |                     ; C27: 2
      |                     ; C28: 2
      |                     ; C29: 2
      |                     ; C30: 2
      |                     ; C31: 2
      |                     ; C33: 2
      |                     ; C34: 2
      |                     ; C35: 2
      |                     ; C36: 2
      |                     ; C40: 2
      |                     ; C41: 2
      |                     ; C42: 2
      |                     ; C43: 2
      |                     ; C44: 2
      |                     ; C45: 2
      |                     ; C46: 2
      |                     ; C47: 2
      |                     ; C48: 2
      |                     ; D2: 2(A)
      |                     ; PV1: -
      |                     ; P_CHG: N
      |                     ; P_COUT: N
      |                     ; P_CTMR: N
      |                     ; P_D1: A
      |                     ; P_R3: 2
      |                     ; P_R8: 2
      |                     ; P_RSHDN_PD: 2
      |                     ; P_U1: GND
      |                     ; Q2: 3(S)
      |                     ; Q3: 1(S1), 4(S2)
      |                     ; R1: 2(n)
      |                     ; R18: 2
      |                     ; R21: 2
      |                     ; R24: 2
      |                     ; R35: 2
      |                     ; R42: 2
      |                     ; R44: 2
      |                     ; R48: 2
      |                     ; U1: 8(CH7), 9(DGND), 14(AGND)
      |                     ; U2: 2(GND), 3(REF2), 4(RESERVED_GND)
      |                     ; U3: 2(GND), 3(REF2), 4(RESERVED_GND)
      |                     ; U4: 3(GND)
      |                     ; U5: 3(GND)
      |                     ; U6: 3(GND)
      |                     ; U7: 3(GND), 8(GND), 13(GND), 18(GND), 23(GND), 28(GND), 33(AGND), 38(GND)
      |                     ; U9: 4(VEE)
      |                     ; U10: 1(GNDP), 2(GNDP), 5(GNDP), 8(GNDP), 9(GNDP), 10(GNDP), 11(GNDP), 12(GNDP), 13(GNDP), 14(GNDP), 15(GNDP), 16(GNDP), 17(GNDP), 18(GNDP)
      |                     ; U11: 2(GND)
      |                     ; U12: 2(GND)
      | 接続部品数　　　　　; 72部品（部品番号で集計。同一ネット全体）
      | 接続端子数　　　　　; 99端子（423端子の部品対応表で集計。ラベル・境界ポートの重複は含めない）
      | この場所の端子数　　; 1端子／1部品（同名ラベルによる接続を除く）
      | 同階層同名ラベル数　; 75個（このラベル自身を含む）
      | 全階層の接続ラベル　; 87個（実際に同じノードへつながるラベル。名前が違う別名も含む）
      | 接続ルール　　　　　; 同じ階層の同じラベル名を仮想配線として結ぶ。別のSubsystem内とは名前だけでつながらず、明示的なConnection Portと配線をたどる。色は用途の表示であり接続を決めない。
      | 確認の範囲　　　　　; 現在の保存回路の端子・配線から求めた静的接続。抵抗やICの内部を導線として短絡せずに集計した。説明の更新は動作シミュレーション、タイミング、実部品の性能・実機動作を保証するものではない。
      | 記録の基準　　　　　; measurement_label_layout_20261022_r01/after_layout_graph.json。部品対応表は端子名の対応付けにのみ使用。
      | 
      | 【この説明欄の略語・記号】
      | 用語1　　　　　　　 ; DC：Direct Current（直流）。ここでは直流電源または直流成分。DCバイアスはコンデンサに重なる直流電圧を指す。
      | 用語2　　　　　　　 ; DC/DC：DC-to-DC Converter（直流電圧変換器）。直流入力を別の直流電圧へ変換する電源回路。絶縁の有無は個々の部品説明で確認する。
      | 用語3　　　　　　　 ; ADC：Analog-to-Digital Converter（アナログ・デジタル変換器）。測定電圧をデジタル値へ変換する回路。電流や温度も、センサーで電圧へ変換した後に読み取る。
      | 用語4　　　　　　　 ; IC：Integrated Circuit（集積回路）。複数の電子素子と機能を小さな半導体チップに集積した部品。
      | 用語5　　　　　　　 ; PWM：Pulse Width Modulation（パルス幅変調）。周期に対するON時間の割合を変えて、スイッチの平均的な電力伝達を調整する方式。
      | 用語6　　　　　　　 ; CH：Channel（測定チャネル）。CH0〜CH7はADCの入力番号であり、同時測定を意味しない。
      | 用語7　　　　　　　 ; MOSFET：Metal-Oxide-Semiconductor Field-Effect Transistor（金属・酸化膜・半導体構造の電界効果トランジスタ）。ゲートとソースの電圧でドレインとソースの導通を制御する素子。N-MOSはNチャネル型を表す。
      | 用語8　　　　　　　 ; LED：Light-Emitting Diode（発光ダイオード）。本回路のゲートドライバ入力では光によって信号を伝え、入力側と出力側を絶縁するために用いる。
      | 用語9　　　　　　　 ; LiFePO4：Lithium Iron Phosphate（リン酸鉄リチウム）。電池の正極材料を示す化学式。英語の頭文字を並べた略語ではない。
      | 用語10　　　　　　　; GND：Ground（回路の基準電位・電流帰路）。この図の共通基準。保護接地や大地への接続を意味するとは限らない。
      | 用語11　　　　　　　; AGND：Analog Ground（アナログ回路の基準端子）。アナログ部分の電流帰路。現図では共通GNDへ接続されるが、実装時の電流経路への配慮は別途必要。
      | 用語12　　　　　　　; DGND：Digital Ground（デジタル回路の基準端子）。デジタル部分の電流帰路。現図では共通GNDへ接続される。
      | 用語13　　　　　　　; VREF/REF：基準電圧を表す端子名。REFはReference（基準）の意味。ADCの変換尺度や電流アンプの出力基準に使う。REF1/REF2の接続電位は個別に確認する。
      | 用語14　　　　　　　; VCC/VDD/VEE/VS：ICの電源端子名。文字の歴史的な由来を現在の接続機能へ当てはめない。現回路のVEEはU8/U10では浮動基準SW、U9ではGND。各電圧・基準は端子と接続を参照する。
      | 用語15　　　　　　　; GNDP：U10の一次側電源の基準端子。絶縁電源の入力側GND。二次側基準VEE=SWと直接同一の導体ではない。
      | 用語16　　　　　　　; SW：Switching Node（スイッチング点）。主電力段の上下MOSFETとL1がつながる、電圧が高速に切り替わる点。GNDとは別電位。
  GND_Label_050 : ConnectionLabel  Description=|  Label=GND
      | この回路での名前　　; GND
      | 種別　　　　　　　　; ConnectionLabel
      | この回路での役割　　; 電池BT1の負極、太陽電池列の負極、制御・測定・保護回路のGNDを結ぶ共通の帰路。高側駆動の浮動帰路SWとは別のノード。
      | 共通帰路の代表接続　; BT1（充電先の蓄電池／51.2V 100Ah LiFePO4）: -
      |                     ; PV1（直列太陽電池列の負極側パネル／400W panel 1/2）: -
      |                     ; U7（RP2040搭載Pico W／SC0918）: 3(GND), 8(GND), 13(GND), 18(GND), 23(GND), 28(GND), 33(AGND), 38(GND)
      |                     ; U1（外付けADC／MCP3208-CI/SL）: 8(CH7), 9(DGND), 14(AGND)
      |                     ; P_U1（保護MOSFETを制御する保護IC／LTC4364IMS-1#PBF）: GND
      |                     ; Q2（同期整流降圧回路の下側スイッチ／TK9R6E15Q5,S1X）: 3(S)
      |                     ; U9（低側の光ゲートドライバ／ACPL-P346-560E）: 4(VEE)
      |                     ; U10（高側ゲート用の浮動電源を作る絶縁DC/DC／UCC14131QDWNRQ1）: 1(GNDP), 2(GNDP), 5(GNDP), 8(GNDP), 9(GNDP), 10(GNDP), 11(GNDP), 12(GNDP), 13(GNDP), 14(GNDP), 15(GNDP), 16(GNDP), 17(GNDP), 18(GNDP)
      | この場所の直接接続　; Q3（RP2040のPWM_Lを受け、U9の入力LED電流をGNDへ引き込む／dual 30V logic-level LED sink）: 4(S2)
      | 直接接続の範囲　　　; このラベルから実際の線・分岐・明示的な境界端子だけを追った接続。同名ラベルによる離れた場所への接続はこの欄に含めない。
      | 同一ネット全端子　　; BT1: -
      |                     ; C1: 2(n)
      |                     ; C2: 2(n)
      |                     ; C3: 2(n)
      |                     ; C4: 2(n)
      |                     ; C7: 2(n)
      |                     ; C8: 2(n)
      |                     ; C9: 2(n)
      |                     ; C10: 2(n)
      |                     ; C13: 2(n)
      |                     ; C14: 2(n)
      |                     ; C15: 2(n)
      |                     ; C16: 2(n)
      |                     ; C17: 2
      |                     ; C18: 2
      |                     ; C19: 2
      |                     ; C20: 2
      |                     ; C21: 2
      |                     ; C22: 2
      |                     ; C23: 2
      |                     ; C24: 2
      |                     ; C25: 2
      |                     ; C26: 2
      |                     ; C27: 2
      |                     ; C28: 2
      |                     ; C29: 2
      |                     ; C30: 2
      |                     ; C31: 2
      |                     ; C33: 2
      |                     ; C34: 2
      |                     ; C35: 2
      |                     ; C36: 2
      |                     ; C40: 2
      |                     ; C41: 2
      |                     ; C42: 2
      |                     ; C43: 2
      |                     ; C44: 2
      |                     ; C45: 2
      |                     ; C46: 2
      |                     ; C47: 2
      |                     ; C48: 2
      |                     ; D2: 2(A)
      |                     ; PV1: -
      |                     ; P_CHG: N
      |                     ; P_COUT: N
      |                     ; P_CTMR: N
      |                     ; P_D1: A
      |                     ; P_R3: 2
      |                     ; P_R8: 2
      |                     ; P_RSHDN_PD: 2
      |                     ; P_U1: GND
      |                     ; Q2: 3(S)
      |                     ; Q3: 1(S1), 4(S2)
      |                     ; R1: 2(n)
      |                     ; R18: 2
      |                     ; R21: 2
      |                     ; R24: 2
      |                     ; R35: 2
      |                     ; R42: 2
      |                     ; R44: 2
      |                     ; R48: 2
      |                     ; U1: 8(CH7), 9(DGND), 14(AGND)
      |                     ; U2: 2(GND), 3(REF2), 4(RESERVED_GND)
      |                     ; U3: 2(GND), 3(REF2), 4(RESERVED_GND)
      |                     ; U4: 3(GND)
      |                     ; U5: 3(GND)
      |                     ; U6: 3(GND)
      |                     ; U7: 3(GND), 8(GND), 13(GND), 18(GND), 23(GND), 28(GND), 33(AGND), 38(GND)
      |                     ; U9: 4(VEE)
      |                     ; U10: 1(GNDP), 2(GNDP), 5(GNDP), 8(GNDP), 9(GNDP), 10(GNDP), 11(GNDP), 12(GNDP), 13(GNDP), 14(GNDP), 15(GNDP), 16(GNDP), 17(GNDP), 18(GNDP)
      |                     ; U11: 2(GND)
      |                     ; U12: 2(GND)
      | 接続部品数　　　　　; 72部品（部品番号で集計。同一ネット全体）
      | 接続端子数　　　　　; 99端子（423端子の部品対応表で集計。ラベル・境界ポートの重複は含めない）
      | この場所の端子数　　; 1端子／1部品（同名ラベルによる接続を除く）
      | 同階層同名ラベル数　; 75個（このラベル自身を含む）
      | 全階層の接続ラベル　; 87個（実際に同じノードへつながるラベル。名前が違う別名も含む）
      | 接続ルール　　　　　; 同じ階層の同じラベル名を仮想配線として結ぶ。別のSubsystem内とは名前だけでつながらず、明示的なConnection Portと配線をたどる。色は用途の表示であり接続を決めない。
      | 確認の範囲　　　　　; 現在の保存回路の端子・配線から求めた静的接続。抵抗やICの内部を導線として短絡せずに集計した。説明の更新は動作シミュレーション、タイミング、実部品の性能・実機動作を保証するものではない。
      | 記録の基準　　　　　; measurement_label_layout_20261022_r01/after_layout_graph.json。部品対応表は端子名の対応付けにのみ使用。
      | 
      | 【この説明欄の略語・記号】
      | 用語1　　　　　　　 ; DC：Direct Current（直流）。ここでは直流電源または直流成分。DCバイアスはコンデンサに重なる直流電圧を指す。
      | 用語2　　　　　　　 ; DC/DC：DC-to-DC Converter（直流電圧変換器）。直流入力を別の直流電圧へ変換する電源回路。絶縁の有無は個々の部品説明で確認する。
      | 用語3　　　　　　　 ; ADC：Analog-to-Digital Converter（アナログ・デジタル変換器）。測定電圧をデジタル値へ変換する回路。電流や温度も、センサーで電圧へ変換した後に読み取る。
      | 用語4　　　　　　　 ; IC：Integrated Circuit（集積回路）。複数の電子素子と機能を小さな半導体チップに集積した部品。
      | 用語5　　　　　　　 ; PWM：Pulse Width Modulation（パルス幅変調）。周期に対するON時間の割合を変えて、スイッチの平均的な電力伝達を調整する方式。
      | 用語6　　　　　　　 ; CH：Channel（測定チャネル）。CH0〜CH7はADCの入力番号であり、同時測定を意味しない。
      | 用語7　　　　　　　 ; MOSFET：Metal-Oxide-Semiconductor Field-Effect Transistor（金属・酸化膜・半導体構造の電界効果トランジスタ）。ゲートとソースの電圧でドレインとソースの導通を制御する素子。N-MOSはNチャネル型を表す。
      | 用語8　　　　　　　 ; LED：Light-Emitting Diode（発光ダイオード）。本回路のゲートドライバ入力では光によって信号を伝え、入力側と出力側を絶縁するために用いる。
      | 用語9　　　　　　　 ; LiFePO4：Lithium Iron Phosphate（リン酸鉄リチウム）。電池の正極材料を示す化学式。英語の頭文字を並べた略語ではない。
      | 用語10　　　　　　　; GND：Ground（回路の基準電位・電流帰路）。この図の共通基準。保護接地や大地への接続を意味するとは限らない。
      | 用語11　　　　　　　; AGND：Analog Ground（アナログ回路の基準端子）。アナログ部分の電流帰路。現図では共通GNDへ接続されるが、実装時の電流経路への配慮は別途必要。
      | 用語12　　　　　　　; DGND：Digital Ground（デジタル回路の基準端子）。デジタル部分の電流帰路。現図では共通GNDへ接続される。
      | 用語13　　　　　　　; VREF/REF：基準電圧を表す端子名。REFはReference（基準）の意味。ADCの変換尺度や電流アンプの出力基準に使う。REF1/REF2の接続電位は個別に確認する。
      | 用語14　　　　　　　; VCC/VDD/VEE/VS：ICの電源端子名。文字の歴史的な由来を現在の接続機能へ当てはめない。現回路のVEEはU8/U10では浮動基準SW、U9ではGND。各電圧・基準は端子と接続を参照する。
      | 用語15　　　　　　　; GNDP：U10の一次側電源の基準端子。絶縁電源の入力側GND。二次側基準VEE=SWと直接同一の導体ではない。
      | 用語16　　　　　　　; SW：Switching Node（スイッチング点）。主電力段の上下MOSFETとL1がつながる、電圧が高速に切り替わる点。GNDとは別電位。
  GND_Label_053 : ConnectionLabel  Description=|  Label=GND
      | この回路での名前　　; GND
      | 種別　　　　　　　　; ConnectionLabel
      | この回路での役割　　; 電池BT1の負極、太陽電池列の負極、制御・測定・保護回路のGNDを結ぶ共通の帰路。高側駆動の浮動帰路SWとは別のノード。
      | 共通帰路の代表接続　; BT1（充電先の蓄電池／51.2V 100Ah LiFePO4）: -
      |                     ; PV1（直列太陽電池列の負極側パネル／400W panel 1/2）: -
      |                     ; U7（RP2040搭載Pico W／SC0918）: 3(GND), 8(GND), 13(GND), 18(GND), 23(GND), 28(GND), 33(AGND), 38(GND)
      |                     ; U1（外付けADC／MCP3208-CI/SL）: 8(CH7), 9(DGND), 14(AGND)
      |                     ; P_U1（保護MOSFETを制御する保護IC／LTC4364IMS-1#PBF）: GND
      |                     ; Q2（同期整流降圧回路の下側スイッチ／TK9R6E15Q5,S1X）: 3(S)
      |                     ; U9（低側の光ゲートドライバ／ACPL-P346-560E）: 4(VEE)
      |                     ; U10（高側ゲート用の浮動電源を作る絶縁DC/DC／UCC14131QDWNRQ1）: 1(GNDP), 2(GNDP), 5(GNDP), 8(GNDP), 9(GNDP), 10(GNDP), 11(GNDP), 12(GNDP), 13(GNDP), 14(GNDP), 15(GNDP), 16(GNDP), 17(GNDP), 18(GNDP)
      | この場所の直接接続　; R1（VIN–GND間へ常時接続し、入力側コンデンサの電荷を徐々に放電する／15 kohm）: 2(n)
      | 直接接続の範囲　　　; このラベルから実際の線・分岐・明示的な境界端子だけを追った接続。同名ラベルによる離れた場所への接続はこの欄に含めない。
      | 同一ネット全端子　　; BT1: -
      |                     ; C1: 2(n)
      |                     ; C2: 2(n)
      |                     ; C3: 2(n)
      |                     ; C4: 2(n)
      |                     ; C7: 2(n)
      |                     ; C8: 2(n)
      |                     ; C9: 2(n)
      |                     ; C10: 2(n)
      |                     ; C13: 2(n)
      |                     ; C14: 2(n)
      |                     ; C15: 2(n)
      |                     ; C16: 2(n)
      |                     ; C17: 2
      |                     ; C18: 2
      |                     ; C19: 2
      |                     ; C20: 2
      |                     ; C21: 2
      |                     ; C22: 2
      |                     ; C23: 2
      |                     ; C24: 2
      |                     ; C25: 2
      |                     ; C26: 2
      |                     ; C27: 2
      |                     ; C28: 2
      |                     ; C29: 2
      |                     ; C30: 2
      |                     ; C31: 2
      |                     ; C33: 2
      |                     ; C34: 2
      |                     ; C35: 2
      |                     ; C36: 2
      |                     ; C40: 2
      |                     ; C41: 2
      |                     ; C42: 2
      |                     ; C43: 2
      |                     ; C44: 2
      |                     ; C45: 2
      |                     ; C46: 2
      |                     ; C47: 2
      |                     ; C48: 2
      |                     ; D2: 2(A)
      |                     ; PV1: -
      |                     ; P_CHG: N
      |                     ; P_COUT: N
      |                     ; P_CTMR: N
      |                     ; P_D1: A
      |                     ; P_R3: 2
      |                     ; P_R8: 2
      |                     ; P_RSHDN_PD: 2
      |                     ; P_U1: GND
      |                     ; Q2: 3(S)
      |                     ; Q3: 1(S1), 4(S2)
      |                     ; R1: 2(n)
      |                     ; R18: 2
      |                     ; R21: 2
      |                     ; R24: 2
      |                     ; R35: 2
      |                     ; R42: 2
      |                     ; R44: 2
      |                     ; R48: 2
      |                     ; U1: 8(CH7), 9(DGND), 14(AGND)
      |                     ; U2: 2(GND), 3(REF2), 4(RESERVED_GND)
      |                     ; U3: 2(GND), 3(REF2), 4(RESERVED_GND)
      |                     ; U4: 3(GND)
      |                     ; U5: 3(GND)
      |                     ; U6: 3(GND)
      |                     ; U7: 3(GND), 8(GND), 13(GND), 18(GND), 23(GND), 28(GND), 33(AGND), 38(GND)
      |                     ; U9: 4(VEE)
      |                     ; U10: 1(GNDP), 2(GNDP), 5(GNDP), 8(GNDP), 9(GNDP), 10(GNDP), 11(GNDP), 12(GNDP), 13(GNDP), 14(GNDP), 15(GNDP), 16(GNDP), 17(GNDP), 18(GNDP)
      |                     ; U11: 2(GND)
      |                     ; U12: 2(GND)
      | 接続部品数　　　　　; 72部品（部品番号で集計。同一ネット全体）
      | 接続端子数　　　　　; 99端子（423端子の部品対応表で集計。ラベル・境界ポートの重複は含めない）
      | この場所の端子数　　; 1端子／1部品（同名ラベルによる接続を除く）
      | 同階層同名ラベル数　; 75個（このラベル自身を含む）
      | 全階層の接続ラベル　; 87個（実際に同じノードへつながるラベル。名前が違う別名も含む）
      | 接続ルール　　　　　; 同じ階層の同じラベル名を仮想配線として結ぶ。別のSubsystem内とは名前だけでつながらず、明示的なConnection Portと配線をたどる。色は用途の表示であり接続を決めない。
      | 確認の範囲　　　　　; 現在の保存回路の端子・配線から求めた静的接続。抵抗やICの内部を導線として短絡せずに集計した。説明の更新は動作シミュレーション、タイミング、実部品の性能・実機動作を保証するものではない。
      | 記録の基準　　　　　; measurement_label_layout_20261022_r01/after_layout_graph.json。部品対応表は端子名の対応付けにのみ使用。
      | 
      | 【この説明欄の略語・記号】
      | 用語1　　　　　　　 ; DC：Direct Current（直流）。ここでは直流電源または直流成分。DCバイアスはコンデンサに重なる直流電圧を指す。
      | 用語2　　　　　　　 ; DC/DC：DC-to-DC Converter（直流電圧変換器）。直流入力を別の直流電圧へ変換する電源回路。絶縁の有無は個々の部品説明で確認する。
      | 用語3　　　　　　　 ; ADC：Analog-to-Digital Converter（アナログ・デジタル変換器）。測定電圧をデジタル値へ変換する回路。電流や温度も、センサーで電圧へ変換した後に読み取る。
      | 用語4　　　　　　　 ; IC：Integrated Circuit（集積回路）。複数の電子素子と機能を小さな半導体チップに集積した部品。
      | 用語5　　　　　　　 ; CH：Channel（測定チャネル）。CH0〜CH7はADCの入力番号であり、同時測定を意味しない。
      | 用語6　　　　　　　 ; MOSFET：Metal-Oxide-Semiconductor Field-Effect Transistor（金属・酸化膜・半導体構造の電界効果トランジスタ）。ゲートとソースの電圧でドレインとソースの導通を制御する素子。N-MOSはNチャネル型を表す。
      | 用語7　　　　　　　 ; LiFePO4：Lithium Iron Phosphate（リン酸鉄リチウム）。電池の正極材料を示す化学式。英語の頭文字を並べた略語ではない。
      | 用語8　　　　　　　 ; GND：Ground（回路の基準電位・電流帰路）。この図の共通基準。保護接地や大地への接続を意味するとは限らない。
      | 用語9　　　　　　　 ; AGND：Analog Ground（アナログ回路の基準端子）。アナログ部分の電流帰路。現図では共通GNDへ接続されるが、実装時の電流経路への配慮は別途必要。
      | 用語10　　　　　　　; DGND：Digital Ground（デジタル回路の基準端子）。デジタル部分の電流帰路。現図では共通GNDへ接続される。
      | 用語11　　　　　　　; VIN/VOUT：入力電圧・出力電圧を表す端子／ネット名。INは入力、OUTは出力。電源変換器の電力端子なのか、検出用端子なのかは対象部品によって異なるため、端子と接続の説明に従う。
      | 用語12　　　　　　　; VREF/REF：基準電圧を表す端子名。REFはReference（基準）の意味。ADCの変換尺度や電流アンプの出力基準に使う。REF1/REF2の接続電位は個別に確認する。
      | 用語13　　　　　　　; VCC/VDD/VEE/VS：ICの電源端子名。文字の歴史的な由来を現在の接続機能へ当てはめない。現回路のVEEはU8/U10では浮動基準SW、U9ではGND。各電圧・基準は端子と接続を参照する。
      | 用語14　　　　　　　; GNDP：U10の一次側電源の基準端子。絶縁電源の入力側GND。二次側基準VEE=SWと直接同一の導体ではない。
      | 用語15　　　　　　　; SW：Switching Node（スイッチング点）。主電力段の上下MOSFETとL1がつながる、電圧が高速に切り替わる点。GNDとは別電位。
  GND_Label_054 : ConnectionLabel  Description=|  Label=GND
      | この回路での名前　　; GND
      | 種別　　　　　　　　; ConnectionLabel
      | この回路での役割　　; 電池BT1の負極、太陽電池列の負極、制御・測定・保護回路のGNDを結ぶ共通の帰路。高側駆動の浮動帰路SWとは別のノード。
      | 共通帰路の代表接続　; BT1（充電先の蓄電池／51.2V 100Ah LiFePO4）: -
      |                     ; PV1（直列太陽電池列の負極側パネル／400W panel 1/2）: -
      |                     ; U7（RP2040搭載Pico W／SC0918）: 3(GND), 8(GND), 13(GND), 18(GND), 23(GND), 28(GND), 33(AGND), 38(GND)
      |                     ; U1（外付けADC／MCP3208-CI/SL）: 8(CH7), 9(DGND), 14(AGND)
      |                     ; P_U1（保護MOSFETを制御する保護IC／LTC4364IMS-1#PBF）: GND
      |                     ; Q2（同期整流降圧回路の下側スイッチ／TK9R6E15Q5,S1X）: 3(S)
      |                     ; U9（低側の光ゲートドライバ／ACPL-P346-560E）: 4(VEE)
      |                     ; U10（高側ゲート用の浮動電源を作る絶縁DC/DC／UCC14131QDWNRQ1）: 1(GNDP), 2(GNDP), 5(GNDP), 8(GNDP), 9(GNDP), 10(GNDP), 11(GNDP), 12(GNDP), 13(GNDP), 14(GNDP), 15(GNDP), 16(GNDP), 17(GNDP), 18(GNDP)
      | この場所の直接接続　; R18（PV入力電圧の分圧抵抗・下側／3.3 kohm 0.1%）: 2
      | 直接接続の範囲　　　; このラベルから実際の線・分岐・明示的な境界端子だけを追った接続。同名ラベルによる離れた場所への接続はこの欄に含めない。
      | 同一ネット全端子　　; BT1: -
      |                     ; C1: 2(n)
      |                     ; C2: 2(n)
      |                     ; C3: 2(n)
      |                     ; C4: 2(n)
      |                     ; C7: 2(n)
      |                     ; C8: 2(n)
      |                     ; C9: 2(n)
      |                     ; C10: 2(n)
      |                     ; C13: 2(n)
      |                     ; C14: 2(n)
      |                     ; C15: 2(n)
      |                     ; C16: 2(n)
      |                     ; C17: 2
      |                     ; C18: 2
      |                     ; C19: 2
      |                     ; C20: 2
      |                     ; C21: 2
      |                     ; C22: 2
      |                     ; C23: 2
      |                     ; C24: 2
      |                     ; C25: 2
      |                     ; C26: 2
      |                     ; C27: 2
      |                     ; C28: 2
      |                     ; C29: 2
      |                     ; C30: 2
      |                     ; C31: 2
      |                     ; C33: 2
      |                     ; C34: 2
      |                     ; C35: 2
      |                     ; C36: 2
      |                     ; C40: 2
      |                     ; C41: 2
      |                     ; C42: 2
      |                     ; C43: 2
      |                     ; C44: 2
      |                     ; C45: 2
      |                     ; C46: 2
      |                     ; C47: 2
      |                     ; C48: 2
      |                     ; D2: 2(A)
      |                     ; PV1: -
      |                     ; P_CHG: N
      |                     ; P_COUT: N
      |                     ; P_CTMR: N
      |                     ; P_D1: A
      |                     ; P_R3: 2
      |                     ; P_R8: 2
      |                     ; P_RSHDN_PD: 2
      |                     ; P_U1: GND
      |                     ; Q2: 3(S)
      |                     ; Q3: 1(S1), 4(S2)
      |                     ; R1: 2(n)
      |                     ; R18: 2
      |                     ; R21: 2
      |                     ; R24: 2
      |                     ; R35: 2
      |                     ; R42: 2
      |                     ; R44: 2
      |                     ; R48: 2
      |                     ; U1: 8(CH7), 9(DGND), 14(AGND)
      |                     ; U2: 2(GND), 3(REF2), 4(RESERVED_GND)
      |                     ; U3: 2(GND), 3(REF2), 4(RESERVED_GND)
      |                     ; U4: 3(GND)
      |                     ; U5: 3(GND)
      |                     ; U6: 3(GND)
      |                     ; U7: 3(GND), 8(GND), 13(GND), 18(GND), 23(GND), 28(GND), 33(AGND), 38(GND)
      |                     ; U9: 4(VEE)
      |                     ; U10: 1(GNDP), 2(GNDP), 5(GNDP), 8(GNDP), 9(GNDP), 10(GNDP), 11(GNDP), 12(GNDP), 13(GNDP), 14(GNDP), 15(GNDP), 16(GNDP), 17(GNDP), 18(GNDP)
      |                     ; U11: 2(GND)
      |                     ; U12: 2(GND)
      | 接続部品数　　　　　; 72部品（部品番号で集計。同一ネット全体）
      | 接続端子数　　　　　; 99端子（423端子の部品対応表で集計。ラベル・境界ポートの重複は含めない）
      | この場所の端子数　　; 1端子／1部品（同名ラベルによる接続を除く）
      | 同階層同名ラベル数　; 75個（このラベル自身を含む）
      | 全階層の接続ラベル　; 87個（実際に同じノードへつながるラベル。名前が違う別名も含む）
      | 接続ルール　　　　　; 同じ階層の同じラベル名を仮想配線として結ぶ。別のSubsystem内とは名前だけでつながらず、明示的なConnection Portと配線をたどる。色は用途の表示であり接続を決めない。
      | 確認の範囲　　　　　; 現在の保存回路の端子・配線から求めた静的接続。抵抗やICの内部を導線として短絡せずに集計した。説明の更新は動作シミュレーション、タイミング、実部品の性能・実機動作を保証するものではない。
      | 記録の基準　　　　　; measurement_label_layout_20261022_r01/after_layout_graph.json。部品対応表は端子名の対応付けにのみ使用。
      | 
      | 【この説明欄の略語・記号】
      | 用語1　　　　　　　 ; DC：Direct Current（直流）。ここでは直流電源または直流成分。DCバイアスはコンデンサに重なる直流電圧を指す。
      | 用語2　　　　　　　 ; DC/DC：DC-to-DC Converter（直流電圧変換器）。直流入力を別の直流電圧へ変換する電源回路。絶縁の有無は個々の部品説明で確認する。
      | 用語3　　　　　　　 ; ADC：Analog-to-Digital Converter（アナログ・デジタル変換器）。測定電圧をデジタル値へ変換する回路。電流や温度も、センサーで電圧へ変換した後に読み取る。
      | 用語4　　　　　　　 ; IC：Integrated Circuit（集積回路）。複数の電子素子と機能を小さな半導体チップに集積した部品。
      | 用語5　　　　　　　 ; CH：Channel（測定チャネル）。CH0〜CH7はADCの入力番号であり、同時測定を意味しない。
      | 用語6　　　　　　　 ; MOSFET：Metal-Oxide-Semiconductor Field-Effect Transistor（金属・酸化膜・半導体構造の電界効果トランジスタ）。ゲートとソースの電圧でドレインとソースの導通を制御する素子。N-MOSはNチャネル型を表す。
      | 用語7　　　　　　　 ; LiFePO4：Lithium Iron Phosphate（リン酸鉄リチウム）。電池の正極材料を示す化学式。英語の頭文字を並べた略語ではない。
      | 用語8　　　　　　　 ; PV：Photovoltaic（太陽光発電）。光を電気へ変える発電方式。PVを含むネット名は太陽電池側の測定・電力経路を表す。
      | 用語9　　　　　　　 ; GND：Ground（回路の基準電位・電流帰路）。この図の共通基準。保護接地や大地への接続を意味するとは限らない。
      | 用語10　　　　　　　; AGND：Analog Ground（アナログ回路の基準端子）。アナログ部分の電流帰路。現図では共通GNDへ接続されるが、実装時の電流経路への配慮は別途必要。
      | 用語11　　　　　　　; DGND：Digital Ground（デジタル回路の基準端子）。デジタル部分の電流帰路。現図では共通GNDへ接続される。
      | 用語12　　　　　　　; VREF/REF：基準電圧を表す端子名。REFはReference（基準）の意味。ADCの変換尺度や電流アンプの出力基準に使う。REF1/REF2の接続電位は個別に確認する。
      | 用語13　　　　　　　; VCC/VDD/VEE/VS：ICの電源端子名。文字の歴史的な由来を現在の接続機能へ当てはめない。現回路のVEEはU8/U10では浮動基準SW、U9ではGND。各電圧・基準は端子と接続を参照する。
      | 用語14　　　　　　　; GNDP：U10の一次側電源の基準端子。絶縁電源の入力側GND。二次側基準VEE=SWと直接同一の導体ではない。
      | 用語15　　　　　　　; SW：Switching Node（スイッチング点）。主電力段の上下MOSFETとL1がつながる、電圧が高速に切り替わる点。GNDとは別電位。
  GND_Label_055 : ConnectionLabel  Description=|  Label=GND
      | この回路での名前　　; GND
      | 種別　　　　　　　　; ConnectionLabel
      | この回路での役割　　; 電池BT1の負極、太陽電池列の負極、制御・測定・保護回路のGNDを結ぶ共通の帰路。高側駆動の浮動帰路SWとは別のノード。
      | 共通帰路の代表接続　; BT1（充電先の蓄電池／51.2V 100Ah LiFePO4）: -
      |                     ; PV1（直列太陽電池列の負極側パネル／400W panel 1/2）: -
      |                     ; U7（RP2040搭載Pico W／SC0918）: 3(GND), 8(GND), 13(GND), 18(GND), 23(GND), 28(GND), 33(AGND), 38(GND)
      |                     ; U1（外付けADC／MCP3208-CI/SL）: 8(CH7), 9(DGND), 14(AGND)
      |                     ; P_U1（保護MOSFETを制御する保護IC／LTC4364IMS-1#PBF）: GND
      |                     ; Q2（同期整流降圧回路の下側スイッチ／TK9R6E15Q5,S1X）: 3(S)
      |                     ; U9（低側の光ゲートドライバ／ACPL-P346-560E）: 4(VEE)
      |                     ; U10（高側ゲート用の浮動電源を作る絶縁DC/DC／UCC14131QDWNRQ1）: 1(GNDP), 2(GNDP), 5(GNDP), 8(GNDP), 9(GNDP), 10(GNDP), 11(GNDP), 12(GNDP), 13(GNDP), 14(GNDP), 15(GNDP), 16(GNDP), 17(GNDP), 18(GNDP)
      | この場所の直接接続　; R21（出力電圧の分圧抵抗・下側／3.3 kohm 0.1%）: 2
      | 直接接続の範囲　　　; このラベルから実際の線・分岐・明示的な境界端子だけを追った接続。同名ラベルによる離れた場所への接続はこの欄に含めない。
      | 同一ネット全端子　　; BT1: -
      |                     ; C1: 2(n)
      |                     ; C2: 2(n)
      |                     ; C3: 2(n)
      |                     ; C4: 2(n)
      |                     ; C7: 2(n)
      |                     ; C8: 2(n)
      |                     ; C9: 2(n)
      |                     ; C10: 2(n)
      |                     ; C13: 2(n)
      |                     ; C14: 2(n)
      |                     ; C15: 2(n)
      |                     ; C16: 2(n)
      |                     ; C17: 2
      |                     ; C18: 2
      |                     ; C19: 2
      |                     ; C20: 2
      |                     ; C21: 2
      |                     ; C22: 2
      |                     ; C23: 2
      |                     ; C24: 2
      |                     ; C25: 2
      |                     ; C26: 2
      |                     ; C27: 2
      |                     ; C28: 2
      |                     ; C29: 2
      |                     ; C30: 2
      |                     ; C31: 2
      |                     ; C33: 2
      |                     ; C34: 2
      |                     ; C35: 2
      |                     ; C36: 2
      |                     ; C40: 2
      |                     ; C41: 2
      |                     ; C42: 2
      |                     ; C43: 2
      |                     ; C44: 2
      |                     ; C45: 2
      |                     ; C46: 2
      |                     ; C47: 2
      |                     ; C48: 2
      |                     ; D2: 2(A)
      |                     ; PV1: -
      |                     ; P_CHG: N
      |                     ; P_COUT: N
      |                     ; P_CTMR: N
      |                     ; P_D1: A
      |                     ; P_R3: 2
      |                     ; P_R8: 2
      |                     ; P_RSHDN_PD: 2
      |                     ; P_U1: GND
      |                     ; Q2: 3(S)
      |                     ; Q3: 1(S1), 4(S2)
      |                     ; R1: 2(n)
      |                     ; R18: 2
      |                     ; R21: 2
      |                     ; R24: 2
      |                     ; R35: 2
      |                     ; R42: 2
      |                     ; R44: 2
      |                     ; R48: 2
      |                     ; U1: 8(CH7), 9(DGND), 14(AGND)
      |                     ; U2: 2(GND), 3(REF2), 4(RESERVED_GND)
      |                     ; U3: 2(GND), 3(REF2), 4(RESERVED_GND)
      |                     ; U4: 3(GND)
      |                     ; U5: 3(GND)
      |                     ; U6: 3(GND)
      |                     ; U7: 3(GND), 8(GND), 13(GND), 18(GND), 23(GND), 28(GND), 33(AGND), 38(GND)
      |                     ; U9: 4(VEE)
      |                     ; U10: 1(GNDP), 2(GNDP), 5(GNDP), 8(GNDP), 9(GNDP), 10(GNDP), 11(GNDP), 12(GNDP), 13(GNDP), 14(GNDP), 15(GNDP), 16(GNDP), 17(GNDP), 18(GNDP)
      |                     ; U11: 2(GND)
      |                     ; U12: 2(GND)
      | 接続部品数　　　　　; 72部品（部品番号で集計。同一ネット全体）
      | 接続端子数　　　　　; 99端子（423端子の部品対応表で集計。ラベル・境界ポートの重複は含めない）
      | この場所の端子数　　; 1端子／1部品（同名ラベルによる接続を除く）
      | 同階層同名ラベル数　; 75個（このラベル自身を含む）
      | 全階層の接続ラベル　; 87個（実際に同じノードへつながるラベル。名前が違う別名も含む）
      | 接続ルール　　　　　; 同じ階層の同じラベル名を仮想配線として結ぶ。別のSubsystem内とは名前だけでつながらず、明示的なConnection Portと配線をたどる。色は用途の表示であり接続を決めない。
      | 確認の範囲　　　　　; 現在の保存回路の端子・配線から求めた静的接続。抵抗やICの内部を導線として短絡せずに集計した。説明の更新は動作シミュレーション、タイミング、実部品の性能・実機動作を保証するものではない。
      | 記録の基準　　　　　; measurement_label_layout_20261022_r01/after_layout_graph.json。部品対応表は端子名の対応付けにのみ使用。
      | 
      | 【この説明欄の略語・記号】
      | 用語1　　　　　　　 ; DC：Direct Current（直流）。ここでは直流電源または直流成分。DCバイアスはコンデンサに重なる直流電圧を指す。
      | 用語2　　　　　　　 ; DC/DC：DC-to-DC Converter（直流電圧変換器）。直流入力を別の直流電圧へ変換する電源回路。絶縁の有無は個々の部品説明で確認する。
      | 用語3　　　　　　　 ; ADC：Analog-to-Digital Converter（アナログ・デジタル変換器）。測定電圧をデジタル値へ変換する回路。電流や温度も、センサーで電圧へ変換した後に読み取る。
      | 用語4　　　　　　　 ; IC：Integrated Circuit（集積回路）。複数の電子素子と機能を小さな半導体チップに集積した部品。
      | 用語5　　　　　　　 ; CH：Channel（測定チャネル）。CH0〜CH7はADCの入力番号であり、同時測定を意味しない。
      | 用語6　　　　　　　 ; MOSFET：Metal-Oxide-Semiconductor Field-Effect Transistor（金属・酸化膜・半導体構造の電界効果トランジスタ）。ゲートとソースの電圧でドレインとソースの導通を制御する素子。N-MOSはNチャネル型を表す。
      | 用語7　　　　　　　 ; LiFePO4：Lithium Iron Phosphate（リン酸鉄リチウム）。電池の正極材料を示す化学式。英語の頭文字を並べた略語ではない。
      | 用語8　　　　　　　 ; GND：Ground（回路の基準電位・電流帰路）。この図の共通基準。保護接地や大地への接続を意味するとは限らない。
      | 用語9　　　　　　　 ; AGND：Analog Ground（アナログ回路の基準端子）。アナログ部分の電流帰路。現図では共通GNDへ接続されるが、実装時の電流経路への配慮は別途必要。
      | 用語10　　　　　　　; DGND：Digital Ground（デジタル回路の基準端子）。デジタル部分の電流帰路。現図では共通GNDへ接続される。
      | 用語11　　　　　　　; VREF/REF：基準電圧を表す端子名。REFはReference（基準）の意味。ADCの変換尺度や電流アンプの出力基準に使う。REF1/REF2の接続電位は個別に確認する。
      | 用語12　　　　　　　; VCC/VDD/VEE/VS：ICの電源端子名。文字の歴史的な由来を現在の接続機能へ当てはめない。現回路のVEEはU8/U10では浮動基準SW、U9ではGND。各電圧・基準は端子と接続を参照する。
      | 用語13　　　　　　　; GNDP：U10の一次側電源の基準端子。絶縁電源の入力側GND。二次側基準VEE=SWと直接同一の導体ではない。
      | 用語14　　　　　　　; SW：Switching Node（スイッチング点）。主電力段の上下MOSFETとL1がつながる、電圧が高速に切り替わる点。GNDとは別電位。
  GND_Label_056 : ConnectionLabel  Description=|  Label=GND
      | この回路での名前　　; GND
      | 種別　　　　　　　　; ConnectionLabel
      | この回路での役割　　; 電池BT1の負極、太陽電池列の負極、制御・測定・保護回路のGNDを結ぶ共通の帰路。高側駆動の浮動帰路SWとは別のノード。
      | 共通帰路の代表接続　; BT1（充電先の蓄電池／51.2V 100Ah LiFePO4）: -
      |                     ; PV1（直列太陽電池列の負極側パネル／400W panel 1/2）: -
      |                     ; U7（RP2040搭載Pico W／SC0918）: 3(GND), 8(GND), 13(GND), 18(GND), 23(GND), 28(GND), 33(AGND), 38(GND)
      |                     ; U1（外付けADC／MCP3208-CI/SL）: 8(CH7), 9(DGND), 14(AGND)
      |                     ; P_U1（保護MOSFETを制御する保護IC／LTC4364IMS-1#PBF）: GND
      |                     ; Q2（同期整流降圧回路の下側スイッチ／TK9R6E15Q5,S1X）: 3(S)
      |                     ; U9（低側の光ゲートドライバ／ACPL-P346-560E）: 4(VEE)
      |                     ; U10（高側ゲート用の浮動電源を作る絶縁DC/DC／UCC14131QDWNRQ1）: 1(GNDP), 2(GNDP), 5(GNDP), 8(GNDP), 9(GNDP), 10(GNDP), 11(GNDP), 12(GNDP), 13(GNDP), 14(GNDP), 15(GNDP), 16(GNDP), 17(GNDP), 18(GNDP)
      | この場所の直接接続　; R24（電池側電圧の分圧抵抗・下側／3.3 kohm 0.1%）: 2
      | 直接接続の範囲　　　; このラベルから実際の線・分岐・明示的な境界端子だけを追った接続。同名ラベルによる離れた場所への接続はこの欄に含めない。
      | 同一ネット全端子　　; BT1: -
      |                     ; C1: 2(n)
      |                     ; C2: 2(n)
      |                     ; C3: 2(n)
      |                     ; C4: 2(n)
      |                     ; C7: 2(n)
      |                     ; C8: 2(n)
      |                     ; C9: 2(n)
      |                     ; C10: 2(n)
      |                     ; C13: 2(n)
      |                     ; C14: 2(n)
      |                     ; C15: 2(n)
      |                     ; C16: 2(n)
      |                     ; C17: 2
      |                     ; C18: 2
      |                     ; C19: 2
      |                     ; C20: 2
      |                     ; C21: 2
      |                     ; C22: 2
      |                     ; C23: 2
      |                     ; C24: 2
      |                     ; C25: 2
      |                     ; C26: 2
      |                     ; C27: 2
      |                     ; C28: 2
      |                     ; C29: 2
      |                     ; C30: 2
      |                     ; C31: 2
      |                     ; C33: 2
      |                     ; C34: 2
      |                     ; C35: 2
      |                     ; C36: 2
      |                     ; C40: 2
      |                     ; C41: 2
      |                     ; C42: 2
      |                     ; C43: 2
      |                     ; C44: 2
      |                     ; C45: 2
      |                     ; C46: 2
      |                     ; C47: 2
      |                     ; C48: 2
      |                     ; D2: 2(A)
      |                     ; PV1: -
      |                     ; P_CHG: N
      |                     ; P_COUT: N
      |                     ; P_CTMR: N
      |                     ; P_D1: A
      |                     ; P_R3: 2
      |                     ; P_R8: 2
      |                     ; P_RSHDN_PD: 2
      |                     ; P_U1: GND
      |                     ; Q2: 3(S)
      |                     ; Q3: 1(S1), 4(S2)
      |                     ; R1: 2(n)
      |                     ; R18: 2
      |                     ; R21: 2
      |                     ; R24: 2
      |                     ; R35: 2
      |                     ; R42: 2
      |                     ; R44: 2
      |                     ; R48: 2
      |                     ; U1: 8(CH7), 9(DGND), 14(AGND)
      |                     ; U2: 2(GND), 3(REF2), 4(RESERVED_GND)
      |                     ; U3: 2(GND), 3(REF2), 4(RESERVED_GND)
      |                     ; U4: 3(GND)
      |                     ; U5: 3(GND)
      |                     ; U6: 3(GND)
      |                     ; U7: 3(GND), 8(GND), 13(GND), 18(GND), 23(GND), 28(GND), 33(AGND), 38(GND)
      |                     ; U9: 4(VEE)
      |                     ; U10: 1(GNDP), 2(GNDP), 5(GNDP), 8(GNDP), 9(GNDP), 10(GNDP), 11(GNDP), 12(GNDP), 13(GNDP), 14(GNDP), 15(GNDP), 16(GNDP), 17(GNDP), 18(GNDP)
      |                     ; U11: 2(GND)
      |                     ; U12: 2(GND)
      | 接続部品数　　　　　; 72部品（部品番号で集計。同一ネット全体）
      | 接続端子数　　　　　; 99端子（423端子の部品対応表で集計。ラベル・境界ポートの重複は含めない）
      | この場所の端子数　　; 1端子／1部品（同名ラベルによる接続を除く）
      | 同階層同名ラベル数　; 75個（このラベル自身を含む）
      | 全階層の接続ラベル　; 87個（実際に同じノードへつながるラベル。名前が違う別名も含む）
      | 接続ルール　　　　　; 同じ階層の同じラベル名を仮想配線として結ぶ。別のSubsystem内とは名前だけでつながらず、明示的なConnection Portと配線をたどる。色は用途の表示であり接続を決めない。
      | 確認の範囲　　　　　; 現在の保存回路の端子・配線から求めた静的接続。抵抗やICの内部を導線として短絡せずに集計した。説明の更新は動作シミュレーション、タイミング、実部品の性能・実機動作を保証するものではない。
      | 記録の基準　　　　　; measurement_label_layout_20261022_r01/after_layout_graph.json。部品対応表は端子名の対応付けにのみ使用。
      | 
      | 【この説明欄の略語・記号】
      | 用語1　　　　　　　 ; DC：Direct Current（直流）。ここでは直流電源または直流成分。DCバイアスはコンデンサに重なる直流電圧を指す。
      | 用語2　　　　　　　 ; DC/DC：DC-to-DC Converter（直流電圧変換器）。直流入力を別の直流電圧へ変換する電源回路。絶縁の有無は個々の部品説明で確認する。
      | 用語3　　　　　　　 ; ADC：Analog-to-Digital Converter（アナログ・デジタル変換器）。測定電圧をデジタル値へ変換する回路。電流や温度も、センサーで電圧へ変換した後に読み取る。
      | 用語4　　　　　　　 ; IC：Integrated Circuit（集積回路）。複数の電子素子と機能を小さな半導体チップに集積した部品。
      | 用語5　　　　　　　 ; CH：Channel（測定チャネル）。CH0〜CH7はADCの入力番号であり、同時測定を意味しない。
      | 用語6　　　　　　　 ; MOSFET：Metal-Oxide-Semiconductor Field-Effect Transistor（金属・酸化膜・半導体構造の電界効果トランジスタ）。ゲートとソースの電圧でドレインとソースの導通を制御する素子。N-MOSはNチャネル型を表す。
      | 用語7　　　　　　　 ; LiFePO4：Lithium Iron Phosphate（リン酸鉄リチウム）。電池の正極材料を示す化学式。英語の頭文字を並べた略語ではない。
      | 用語8　　　　　　　 ; GND：Ground（回路の基準電位・電流帰路）。この図の共通基準。保護接地や大地への接続を意味するとは限らない。
      | 用語9　　　　　　　 ; AGND：Analog Ground（アナログ回路の基準端子）。アナログ部分の電流帰路。現図では共通GNDへ接続されるが、実装時の電流経路への配慮は別途必要。
      | 用語10　　　　　　　; DGND：Digital Ground（デジタル回路の基準端子）。デジタル部分の電流帰路。現図では共通GNDへ接続される。
      | 用語11　　　　　　　; VREF/REF：基準電圧を表す端子名。REFはReference（基準）の意味。ADCの変換尺度や電流アンプの出力基準に使う。REF1/REF2の接続電位は個別に確認する。
      | 用語12　　　　　　　; VCC/VDD/VEE/VS：ICの電源端子名。文字の歴史的な由来を現在の接続機能へ当てはめない。現回路のVEEはU8/U10では浮動基準SW、U9ではGND。各電圧・基準は端子と接続を参照する。
      | 用語13　　　　　　　; GNDP：U10の一次側電源の基準端子。絶縁電源の入力側GND。二次側基準VEE=SWと直接同一の導体ではない。
      | 用語14　　　　　　　; SW：Switching Node（スイッチング点）。主電力段の上下MOSFETとL1がつながる、電圧が高速に切り替わる点。GNDとは別電位。
  GND_Label_057 : ConnectionLabel  Description=|  Label=GND
      | この回路での名前　　; GND
      | 種別　　　　　　　　; ConnectionLabel
      | この回路での役割　　; 電池BT1の負極、太陽電池列の負極、制御・測定・保護回路のGNDを結ぶ共通の帰路。高側駆動の浮動帰路SWとは別のノード。
      | 共通帰路の代表接続　; BT1（充電先の蓄電池／51.2V 100Ah LiFePO4）: -
      |                     ; PV1（直列太陽電池列の負極側パネル／400W panel 1/2）: -
      |                     ; U7（RP2040搭載Pico W／SC0918）: 3(GND), 8(GND), 13(GND), 18(GND), 23(GND), 28(GND), 33(AGND), 38(GND)
      |                     ; U1（外付けADC／MCP3208-CI/SL）: 8(CH7), 9(DGND), 14(AGND)
      |                     ; P_U1（保護MOSFETを制御する保護IC／LTC4364IMS-1#PBF）: GND
      |                     ; Q2（同期整流降圧回路の下側スイッチ／TK9R6E15Q5,S1X）: 3(S)
      |                     ; U9（低側の光ゲートドライバ／ACPL-P346-560E）: 4(VEE)
      |                     ; U10（高側ゲート用の浮動電源を作る絶縁DC/DC／UCC14131QDWNRQ1）: 1(GNDP), 2(GNDP), 5(GNDP), 8(GNDP), 9(GNDP), 10(GNDP), 11(GNDP), 12(GNDP), 13(GNDP), 14(GNDP), 15(GNDP), 16(GNDP), 17(GNDP), 18(GNDP)
      | この場所の直接接続　; R35（Q3AゲートをGNDへ引き下げ、RP2040未駆動時のLED消灯側の状態を作る／10k 1%）: 2
      | 直接接続の範囲　　　; このラベルから実際の線・分岐・明示的な境界端子だけを追った接続。同名ラベルによる離れた場所への接続はこの欄に含めない。
      | 同一ネット全端子　　; BT1: -
      |                     ; C1: 2(n)
      |                     ; C2: 2(n)
      |                     ; C3: 2(n)
      |                     ; C4: 2(n)
      |                     ; C7: 2(n)
      |                     ; C8: 2(n)
      |                     ; C9: 2(n)
      |                     ; C10: 2(n)
      |                     ; C13: 2(n)
      |                     ; C14: 2(n)
      |                     ; C15: 2(n)
      |                     ; C16: 2(n)
      |                     ; C17: 2
      |                     ; C18: 2
      |                     ; C19: 2
      |                     ; C20: 2
      |                     ; C21: 2
      |                     ; C22: 2
      |                     ; C23: 2
      |                     ; C24: 2
      |                     ; C25: 2
      |                     ; C26: 2
      |                     ; C27: 2
      |                     ; C28: 2
      |                     ; C29: 2
      |                     ; C30: 2
      |                     ; C31: 2
      |                     ; C33: 2
      |                     ; C34: 2
      |                     ; C35: 2
      |                     ; C36: 2
      |                     ; C40: 2
      |                     ; C41: 2
      |                     ; C42: 2
      |                     ; C43: 2
      |                     ; C44: 2
      |                     ; C45: 2
      |                     ; C46: 2
      |                     ; C47: 2
      |                     ; C48: 2
      |                     ; D2: 2(A)
      |                     ; PV1: -
      |                     ; P_CHG: N
      |                     ; P_COUT: N
      |                     ; P_CTMR: N
      |                     ; P_D1: A
      |                     ; P_R3: 2
      |                     ; P_R8: 2
      |                     ; P_RSHDN_PD: 2
      |                     ; P_U1: GND
      |                     ; Q2: 3(S)
      |                     ; Q3: 1(S1), 4(S2)
      |                     ; R1: 2(n)
      |                     ; R18: 2
      |                     ; R21: 2
      |                     ; R24: 2
      |                     ; R35: 2
      |                     ; R42: 2
      |                     ; R44: 2
      |                     ; R48: 2
      |                     ; U1: 8(CH7), 9(DGND), 14(AGND)
      |                     ; U2: 2(GND), 3(REF2), 4(RESERVED_GND)
      |                     ; U3: 2(GND), 3(REF2), 4(RESERVED_GND)
      |                     ; U4: 3(GND)
      |                     ; U5: 3(GND)
      |                     ; U6: 3(GND)
      |                     ; U7: 3(GND), 8(GND), 13(GND), 18(GND), 23(GND), 28(GND), 33(AGND), 38(GND)
      |                     ; U9: 4(VEE)
      |                     ; U10: 1(GNDP), 2(GNDP), 5(GNDP), 8(GNDP), 9(GNDP), 10(GNDP), 11(GNDP), 12(GNDP), 13(GNDP), 14(GNDP), 15(GNDP), 16(GNDP), 17(GNDP), 18(GNDP)
      |                     ; U11: 2(GND)
      |                     ; U12: 2(GND)
      | 接続部品数　　　　　; 72部品（部品番号で集計。同一ネット全体）
      | 接続端子数　　　　　; 99端子（423端子の部品対応表で集計。ラベル・境界ポートの重複は含めない）
      | この場所の端子数　　; 1端子／1部品（同名ラベルによる接続を除く）
      | 同階層同名ラベル数　; 75個（このラベル自身を含む）
      | 全階層の接続ラベル　; 87個（実際に同じノードへつながるラベル。名前が違う別名も含む）
      | 接続ルール　　　　　; 同じ階層の同じラベル名を仮想配線として結ぶ。別のSubsystem内とは名前だけでつながらず、明示的なConnection Portと配線をたどる。色は用途の表示であり接続を決めない。
      | 確認の範囲　　　　　; 現在の保存回路の端子・配線から求めた静的接続。抵抗やICの内部を導線として短絡せずに集計した。説明の更新は動作シミュレーション、タイミング、実部品の性能・実機動作を保証するものではない。
      | 記録の基準　　　　　; measurement_label_layout_20261022_r01/after_layout_graph.json。部品対応表は端子名の対応付けにのみ使用。
      | 
      | 【この説明欄の略語・記号】
      | 用語1　　　　　　　 ; DC：Direct Current（直流）。ここでは直流電源または直流成分。DCバイアスはコンデンサに重なる直流電圧を指す。
      | 用語2　　　　　　　 ; DC/DC：DC-to-DC Converter（直流電圧変換器）。直流入力を別の直流電圧へ変換する電源回路。絶縁の有無は個々の部品説明で確認する。
      | 用語3　　　　　　　 ; ADC：Analog-to-Digital Converter（アナログ・デジタル変換器）。測定電圧をデジタル値へ変換する回路。電流や温度も、センサーで電圧へ変換した後に読み取る。
      | 用語4　　　　　　　 ; IC：Integrated Circuit（集積回路）。複数の電子素子と機能を小さな半導体チップに集積した部品。
      | 用語5　　　　　　　 ; CH：Channel（測定チャネル）。CH0〜CH7はADCの入力番号であり、同時測定を意味しない。
      | 用語6　　　　　　　 ; MOSFET：Metal-Oxide-Semiconductor Field-Effect Transistor（金属・酸化膜・半導体構造の電界効果トランジスタ）。ゲートとソースの電圧でドレインとソースの導通を制御する素子。N-MOSはNチャネル型を表す。
      | 用語7　　　　　　　 ; LED：Light-Emitting Diode（発光ダイオード）。本回路のゲートドライバ入力では光によって信号を伝え、入力側と出力側を絶縁するために用いる。
      | 用語8　　　　　　　 ; LiFePO4：Lithium Iron Phosphate（リン酸鉄リチウム）。電池の正極材料を示す化学式。英語の頭文字を並べた略語ではない。
      | 用語9　　　　　　　 ; GND：Ground（回路の基準電位・電流帰路）。この図の共通基準。保護接地や大地への接続を意味するとは限らない。
      | 用語10　　　　　　　; AGND：Analog Ground（アナログ回路の基準端子）。アナログ部分の電流帰路。現図では共通GNDへ接続されるが、実装時の電流経路への配慮は別途必要。
      | 用語11　　　　　　　; DGND：Digital Ground（デジタル回路の基準端子）。デジタル部分の電流帰路。現図では共通GNDへ接続される。
      | 用語12　　　　　　　; VREF/REF：基準電圧を表す端子名。REFはReference（基準）の意味。ADCの変換尺度や電流アンプの出力基準に使う。REF1/REF2の接続電位は個別に確認する。
      | 用語13　　　　　　　; VCC/VDD/VEE/VS：ICの電源端子名。文字の歴史的な由来を現在の接続機能へ当てはめない。現回路のVEEはU8/U10では浮動基準SW、U9ではGND。各電圧・基準は端子と接続を参照する。
      | 用語14　　　　　　　; GNDP：U10の一次側電源の基準端子。絶縁電源の入力側GND。二次側基準VEE=SWと直接同一の導体ではない。
      | 用語15　　　　　　　; SW：Switching Node（スイッチング点）。主電力段の上下MOSFETとL1がつながる、電圧が高速に切り替わる点。GNDとは別電位。
  GND_Label_058 : ConnectionLabel  Description=|  Label=GND
      | この回路での名前　　; GND
      | 種別　　　　　　　　; ConnectionLabel
      | この回路での役割　　; 電池BT1の負極、太陽電池列の負極、制御・測定・保護回路のGNDを結ぶ共通の帰路。高側駆動の浮動帰路SWとは別のノード。
      | 共通帰路の代表接続　; BT1（充電先の蓄電池／51.2V 100Ah LiFePO4）: -
      |                     ; PV1（直列太陽電池列の負極側パネル／400W panel 1/2）: -
      |                     ; U7（RP2040搭載Pico W／SC0918）: 3(GND), 8(GND), 13(GND), 18(GND), 23(GND), 28(GND), 33(AGND), 38(GND)
      |                     ; U1（外付けADC／MCP3208-CI/SL）: 8(CH7), 9(DGND), 14(AGND)
      |                     ; P_U1（保護MOSFETを制御する保護IC／LTC4364IMS-1#PBF）: GND
      |                     ; Q2（同期整流降圧回路の下側スイッチ／TK9R6E15Q5,S1X）: 3(S)
      |                     ; U9（低側の光ゲートドライバ／ACPL-P346-560E）: 4(VEE)
      |                     ; U10（高側ゲート用の浮動電源を作る絶縁DC/DC／UCC14131QDWNRQ1）: 1(GNDP), 2(GNDP), 5(GNDP), 8(GNDP), 9(GNDP), 10(GNDP), 11(GNDP), 12(GNDP), 13(GNDP), 14(GNDP), 15(GNDP), 16(GNDP), 17(GNDP), 18(GNDP)
      | この場所の直接接続　; R42（Q3BゲートをGNDへ引き下げ、RP2040未駆動時のLED消灯側の状態を作る／10k 1%）: 2
      | 直接接続の範囲　　　; このラベルから実際の線・分岐・明示的な境界端子だけを追った接続。同名ラベルによる離れた場所への接続はこの欄に含めない。
      | 同一ネット全端子　　; BT1: -
      |                     ; C1: 2(n)
      |                     ; C2: 2(n)
      |                     ; C3: 2(n)
      |                     ; C4: 2(n)
      |                     ; C7: 2(n)
      |                     ; C8: 2(n)
      |                     ; C9: 2(n)
      |                     ; C10: 2(n)
      |                     ; C13: 2(n)
      |                     ; C14: 2(n)
      |                     ; C15: 2(n)
      |                     ; C16: 2(n)
      |                     ; C17: 2
      |                     ; C18: 2
      |                     ; C19: 2
      |                     ; C20: 2
      |                     ; C21: 2
      |                     ; C22: 2
      |                     ; C23: 2
      |                     ; C24: 2
      |                     ; C25: 2
      |                     ; C26: 2
      |                     ; C27: 2
      |                     ; C28: 2
      |                     ; C29: 2
      |                     ; C30: 2
      |                     ; C31: 2
      |                     ; C33: 2
      |                     ; C34: 2
      |                     ; C35: 2
      |                     ; C36: 2
      |                     ; C40: 2
      |                     ; C41: 2
      |                     ; C42: 2
      |                     ; C43: 2
      |                     ; C44: 2
      |                     ; C45: 2
      |                     ; C46: 2
      |                     ; C47: 2
      |                     ; C48: 2
      |                     ; D2: 2(A)
      |                     ; PV1: -
      |                     ; P_CHG: N
      |                     ; P_COUT: N
      |                     ; P_CTMR: N
      |                     ; P_D1: A
      |                     ; P_R3: 2
      |                     ; P_R8: 2
      |                     ; P_RSHDN_PD: 2
      |                     ; P_U1: GND
      |                     ; Q2: 3(S)
      |                     ; Q3: 1(S1), 4(S2)
      |                     ; R1: 2(n)
      |                     ; R18: 2
      |                     ; R21: 2
      |                     ; R24: 2
      |                     ; R35: 2
      |                     ; R42: 2
      |                     ; R44: 2
      |                     ; R48: 2
      |                     ; U1: 8(CH7), 9(DGND), 14(AGND)
      |                     ; U2: 2(GND), 3(REF2), 4(RESERVED_GND)
      |                     ; U3: 2(GND), 3(REF2), 4(RESERVED_GND)
      |                     ; U4: 3(GND)
      |                     ; U5: 3(GND)
      |                     ; U6: 3(GND)
      |                     ; U7: 3(GND), 8(GND), 13(GND), 18(GND), 23(GND), 28(GND), 33(AGND), 38(GND)
      |                     ; U9: 4(VEE)
      |                     ; U10: 1(GNDP), 2(GNDP), 5(GNDP), 8(GNDP), 9(GNDP), 10(GNDP), 11(GNDP), 12(GNDP), 13(GNDP), 14(GNDP), 15(GNDP), 16(GNDP), 17(GNDP), 18(GNDP)
      |                     ; U11: 2(GND)
      |                     ; U12: 2(GND)
      | 接続部品数　　　　　; 72部品（部品番号で集計。同一ネット全体）
      | 接続端子数　　　　　; 99端子（423端子の部品対応表で集計。ラベル・境界ポートの重複は含めない）
      | この場所の端子数　　; 1端子／1部品（同名ラベルによる接続を除く）
      | 同階層同名ラベル数　; 75個（このラベル自身を含む）
      | 全階層の接続ラベル　; 87個（実際に同じノードへつながるラベル。名前が違う別名も含む）
      | 接続ルール　　　　　; 同じ階層の同じラベル名を仮想配線として結ぶ。別のSubsystem内とは名前だけでつながらず、明示的なConnection Portと配線をたどる。色は用途の表示であり接続を決めない。
      | 確認の範囲　　　　　; 現在の保存回路の端子・配線から求めた静的接続。抵抗やICの内部を導線として短絡せずに集計した。説明の更新は動作シミュレーション、タイミング、実部品の性能・実機動作を保証するものではない。
      | 記録の基準　　　　　; measurement_label_layout_20261022_r01/after_layout_graph.json。部品対応表は端子名の対応付けにのみ使用。
      | 
      | 【この説明欄の略語・記号】
      | 用語1　　　　　　　 ; DC：Direct Current（直流）。ここでは直流電源または直流成分。DCバイアスはコンデンサに重なる直流電圧を指す。
      | 用語2　　　　　　　 ; DC/DC：DC-to-DC Converter（直流電圧変換器）。直流入力を別の直流電圧へ変換する電源回路。絶縁の有無は個々の部品説明で確認する。
      | 用語3　　　　　　　 ; ADC：Analog-to-Digital Converter（アナログ・デジタル変換器）。測定電圧をデジタル値へ変換する回路。電流や温度も、センサーで電圧へ変換した後に読み取る。
      | 用語4　　　　　　　 ; IC：Integrated Circuit（集積回路）。複数の電子素子と機能を小さな半導体チップに集積した部品。
      | 用語5　　　　　　　 ; CH：Channel（測定チャネル）。CH0〜CH7はADCの入力番号であり、同時測定を意味しない。
      | 用語6　　　　　　　 ; MOSFET：Metal-Oxide-Semiconductor Field-Effect Transistor（金属・酸化膜・半導体構造の電界効果トランジスタ）。ゲートとソースの電圧でドレインとソースの導通を制御する素子。N-MOSはNチャネル型を表す。
      | 用語7　　　　　　　 ; LED：Light-Emitting Diode（発光ダイオード）。本回路のゲートドライバ入力では光によって信号を伝え、入力側と出力側を絶縁するために用いる。
      | 用語8　　　　　　　 ; LiFePO4：Lithium Iron Phosphate（リン酸鉄リチウム）。電池の正極材料を示す化学式。英語の頭文字を並べた略語ではない。
      | 用語9　　　　　　　 ; GND：Ground（回路の基準電位・電流帰路）。この図の共通基準。保護接地や大地への接続を意味するとは限らない。
      | 用語10　　　　　　　; AGND：Analog Ground（アナログ回路の基準端子）。アナログ部分の電流帰路。現図では共通GNDへ接続されるが、実装時の電流経路への配慮は別途必要。
      | 用語11　　　　　　　; DGND：Digital Ground（デジタル回路の基準端子）。デジタル部分の電流帰路。現図では共通GNDへ接続される。
      | 用語12　　　　　　　; VREF/REF：基準電圧を表す端子名。REFはReference（基準）の意味。ADCの変換尺度や電流アンプの出力基準に使う。REF1/REF2の接続電位は個別に確認する。
      | 用語13　　　　　　　; VCC/VDD/VEE/VS：ICの電源端子名。文字の歴史的な由来を現在の接続機能へ当てはめない。現回路のVEEはU8/U10では浮動基準SW、U9ではGND。各電圧・基準は端子と接続を参照する。
      | 用語14　　　　　　　; GNDP：U10の一次側電源の基準端子。絶縁電源の入力側GND。二次側基準VEE=SWと直接同一の導体ではない。
      | 用語15　　　　　　　; SW：Switching Node（スイッチング点）。主電力段の上下MOSFETとL1がつながる、電圧が高速に切り替わる点。GNDとは別電位。
  GND_Label_060 : ConnectionLabel  Description=|  Label=GND
      | この回路での名前　　; GND
      | 種別　　　　　　　　; ConnectionLabel
      | この回路での役割　　; 電池BT1の負極、太陽電池列の負極、制御・測定・保護回路のGNDを結ぶ共通の帰路。高側駆動の浮動帰路SWとは別のノード。
      | 共通帰路の代表接続　; BT1（充電先の蓄電池／51.2V 100Ah LiFePO4）: -
      |                     ; PV1（直列太陽電池列の負極側パネル／400W panel 1/2）: -
      |                     ; U7（RP2040搭載Pico W／SC0918）: 3(GND), 8(GND), 13(GND), 18(GND), 23(GND), 28(GND), 33(AGND), 38(GND)
      |                     ; U1（外付けADC／MCP3208-CI/SL）: 8(CH7), 9(DGND), 14(AGND)
      |                     ; P_U1（保護MOSFETを制御する保護IC／LTC4364IMS-1#PBF）: GND
      |                     ; Q2（同期整流降圧回路の下側スイッチ／TK9R6E15Q5,S1X）: 3(S)
      |                     ; U9（低側の光ゲートドライバ／ACPL-P346-560E）: 4(VEE)
      |                     ; U10（高側ゲート用の浮動電源を作る絶縁DC/DC／UCC14131QDWNRQ1）: 1(GNDP), 2(GNDP), 5(GNDP), 8(GNDP), 9(GNDP), 10(GNDP), 11(GNDP), 12(GNDP), 13(GNDP), 14(GNDP), 15(GNDP), 16(GNDP), 17(GNDP), 18(GNDP)
      | この場所の直接接続　; R48（BIAS_ENをGNDへ引き下げ、RP2040未駆動時のU10停止側の状態を作る／10k 1%）: 2
      | 直接接続の範囲　　　; このラベルから実際の線・分岐・明示的な境界端子だけを追った接続。同名ラベルによる離れた場所への接続はこの欄に含めない。
      | 同一ネット全端子　　; BT1: -
      |                     ; C1: 2(n)
      |                     ; C2: 2(n)
      |                     ; C3: 2(n)
      |                     ; C4: 2(n)
      |                     ; C7: 2(n)
      |                     ; C8: 2(n)
      |                     ; C9: 2(n)
      |                     ; C10: 2(n)
      |                     ; C13: 2(n)
      |                     ; C14: 2(n)
      |                     ; C15: 2(n)
      |                     ; C16: 2(n)
      |                     ; C17: 2
      |                     ; C18: 2
      |                     ; C19: 2
      |                     ; C20: 2
      |                     ; C21: 2
      |                     ; C22: 2
      |                     ; C23: 2
      |                     ; C24: 2
      |                     ; C25: 2
      |                     ; C26: 2
      |                     ; C27: 2
      |                     ; C28: 2
      |                     ; C29: 2
      |                     ; C30: 2
      |                     ; C31: 2
      |                     ; C33: 2
      |                     ; C34: 2
      |                     ; C35: 2
      |                     ; C36: 2
      |                     ; C40: 2
      |                     ; C41: 2
      |                     ; C42: 2
      |                     ; C43: 2
      |                     ; C44: 2
      |                     ; C45: 2
      |                     ; C46: 2
      |                     ; C47: 2
      |                     ; C48: 2
      |                     ; D2: 2(A)
      |                     ; PV1: -
      |                     ; P_CHG: N
      |                     ; P_COUT: N
      |                     ; P_CTMR: N
      |                     ; P_D1: A
      |                     ; P_R3: 2
      |                     ; P_R8: 2
      |                     ; P_RSHDN_PD: 2
      |                     ; P_U1: GND
      |                     ; Q2: 3(S)
      |                     ; Q3: 1(S1), 4(S2)
      |                     ; R1: 2(n)
      |                     ; R18: 2
      |                     ; R21: 2
      |                     ; R24: 2
      |                     ; R35: 2
      |                     ; R42: 2
      |                     ; R44: 2
      |                     ; R48: 2
      |                     ; U1: 8(CH7), 9(DGND), 14(AGND)
      |                     ; U2: 2(GND), 3(REF2), 4(RESERVED_GND)
      |                     ; U3: 2(GND), 3(REF2), 4(RESERVED_GND)
      |                     ; U4: 3(GND)
      |                     ; U5: 3(GND)
      |                     ; U6: 3(GND)
      |                     ; U7: 3(GND), 8(GND), 13(GND), 18(GND), 23(GND), 28(GND), 33(AGND), 38(GND)
      |                     ; U9: 4(VEE)
      |                     ; U10: 1(GNDP), 2(GNDP), 5(GNDP), 8(GNDP), 9(GNDP), 10(GNDP), 11(GNDP), 12(GNDP), 13(GNDP), 14(GNDP), 15(GNDP), 16(GNDP), 17(GNDP), 18(GNDP)
      |                     ; U11: 2(GND)
      |                     ; U12: 2(GND)
      | 接続部品数　　　　　; 72部品（部品番号で集計。同一ネット全体）
      | 接続端子数　　　　　; 99端子（423端子の部品対応表で集計。ラベル・境界ポートの重複は含めない）
      | この場所の端子数　　; 1端子／1部品（同名ラベルによる接続を除く）
      | 同階層同名ラベル数　; 75個（このラベル自身を含む）
      | 全階層の接続ラベル　; 87個（実際に同じノードへつながるラベル。名前が違う別名も含む）
      | 接続ルール　　　　　; 同じ階層の同じラベル名を仮想配線として結ぶ。別のSubsystem内とは名前だけでつながらず、明示的なConnection Portと配線をたどる。色は用途の表示であり接続を決めない。
      | 確認の範囲　　　　　; 現在の保存回路の端子・配線から求めた静的接続。抵抗やICの内部を導線として短絡せずに集計した。説明の更新は動作シミュレーション、タイミング、実部品の性能・実機動作を保証するものではない。
      | 記録の基準　　　　　; measurement_label_layout_20261022_r01/after_layout_graph.json。部品対応表は端子名の対応付けにのみ使用。
      | 
      | 【この説明欄の略語・記号】
      | 用語1　　　　　　　 ; DC：Direct Current（直流）。ここでは直流電源または直流成分。DCバイアスはコンデンサに重なる直流電圧を指す。
      | 用語2　　　　　　　 ; DC/DC：DC-to-DC Converter（直流電圧変換器）。直流入力を別の直流電圧へ変換する電源回路。絶縁の有無は個々の部品説明で確認する。
      | 用語3　　　　　　　 ; ADC：Analog-to-Digital Converter（アナログ・デジタル変換器）。測定電圧をデジタル値へ変換する回路。電流や温度も、センサーで電圧へ変換した後に読み取る。
      | 用語4　　　　　　　 ; IC：Integrated Circuit（集積回路）。複数の電子素子と機能を小さな半導体チップに集積した部品。
      | 用語5　　　　　　　 ; CH：Channel（測定チャネル）。CH0〜CH7はADCの入力番号であり、同時測定を意味しない。
      | 用語6　　　　　　　 ; MOSFET：Metal-Oxide-Semiconductor Field-Effect Transistor（金属・酸化膜・半導体構造の電界効果トランジスタ）。ゲートとソースの電圧でドレインとソースの導通を制御する素子。N-MOSはNチャネル型を表す。
      | 用語7　　　　　　　 ; LiFePO4：Lithium Iron Phosphate（リン酸鉄リチウム）。電池の正極材料を示す化学式。英語の頭文字を並べた略語ではない。
      | 用語8　　　　　　　 ; GND：Ground（回路の基準電位・電流帰路）。この図の共通基準。保護接地や大地への接続を意味するとは限らない。
      | 用語9　　　　　　　 ; AGND：Analog Ground（アナログ回路の基準端子）。アナログ部分の電流帰路。現図では共通GNDへ接続されるが、実装時の電流経路への配慮は別途必要。
      | 用語10　　　　　　　; DGND：Digital Ground（デジタル回路の基準端子）。デジタル部分の電流帰路。現図では共通GNDへ接続される。
      | 用語11　　　　　　　; EN：Enable（動作許可）。対象機能の動作を許可する信号。端子ごとの有効レベルや接続状態に従う。
      | 用語12　　　　　　　; VREF/REF：基準電圧を表す端子名。REFはReference（基準）の意味。ADCの変換尺度や電流アンプの出力基準に使う。REF1/REF2の接続電位は個別に確認する。
      | 用語13　　　　　　　; VCC/VDD/VEE/VS：ICの電源端子名。文字の歴史的な由来を現在の接続機能へ当てはめない。現回路のVEEはU8/U10では浮動基準SW、U9ではGND。各電圧・基準は端子と接続を参照する。
      | 用語14　　　　　　　; GNDP：U10の一次側電源の基準端子。絶縁電源の入力側GND。二次側基準VEE=SWと直接同一の導体ではない。
      | 用語15　　　　　　　; SW：Switching Node（スイッチング点）。主電力段の上下MOSFETとL1がつながる、電圧が高速に切り替わる点。GNDとは別電位。
  GND_Label_064 : ConnectionLabel  Description=|  Label=GND
      | この回路での名前　　; GND
      | 種別　　　　　　　　; ConnectionLabel
      | この回路での役割　　; 電池BT1の負極、太陽電池列の負極、制御・測定・保護回路のGNDを結ぶ共通の帰路。高側駆動の浮動帰路SWとは別のノード。
      | 共通帰路の代表接続　; BT1（充電先の蓄電池／51.2V 100Ah LiFePO4）: -
      |                     ; PV1（直列太陽電池列の負極側パネル／400W panel 1/2）: -
      |                     ; U7（RP2040搭載Pico W／SC0918）: 3(GND), 8(GND), 13(GND), 18(GND), 23(GND), 28(GND), 33(AGND), 38(GND)
      |                     ; U1（外付けADC／MCP3208-CI/SL）: 8(CH7), 9(DGND), 14(AGND)
      |                     ; P_U1（保護MOSFETを制御する保護IC／LTC4364IMS-1#PBF）: GND
      |                     ; Q2（同期整流降圧回路の下側スイッチ／TK9R6E15Q5,S1X）: 3(S)
      |                     ; U9（低側の光ゲートドライバ／ACPL-P346-560E）: 4(VEE)
      |                     ; U10（高側ゲート用の浮動電源を作る絶縁DC/DC／UCC14131QDWNRQ1）: 1(GNDP), 2(GNDP), 5(GNDP), 8(GNDP), 9(GNDP), 10(GNDP), 11(GNDP), 12(GNDP), 13(GNDP), 14(GNDP), 15(GNDP), 16(GNDP), 17(GNDP), 18(GNDP)
      | この場所の直接接続　; U1（外付けADC／MCP3208-CI/SL）: 9(DGND)
      | 直接接続の範囲　　　; このラベルから実際の線・分岐・明示的な境界端子だけを追った接続。同名ラベルによる離れた場所への接続はこの欄に含めない。
      | 同一ネット全端子　　; BT1: -
      |                     ; C1: 2(n)
      |                     ; C2: 2(n)
      |                     ; C3: 2(n)
      |                     ; C4: 2(n)
      |                     ; C7: 2(n)
      |                     ; C8: 2(n)
      |                     ; C9: 2(n)
      |                     ; C10: 2(n)
      |                     ; C13: 2(n)
      |                     ; C14: 2(n)
      |                     ; C15: 2(n)
      |                     ; C16: 2(n)
      |                     ; C17: 2
      |                     ; C18: 2
      |                     ; C19: 2
      |                     ; C20: 2
      |                     ; C21: 2
      |                     ; C22: 2
      |                     ; C23: 2
      |                     ; C24: 2
      |                     ; C25: 2
      |                     ; C26: 2
      |                     ; C27: 2
      |                     ; C28: 2
      |                     ; C29: 2
      |                     ; C30: 2
      |                     ; C31: 2
      |                     ; C33: 2
      |                     ; C34: 2
      |                     ; C35: 2
      |                     ; C36: 2
      |                     ; C40: 2
      |                     ; C41: 2
      |                     ; C42: 2
      |                     ; C43: 2
      |                     ; C44: 2
      |                     ; C45: 2
      |                     ; C46: 2
      |                     ; C47: 2
      |                     ; C48: 2
      |                     ; D2: 2(A)
      |                     ; PV1: -
      |                     ; P_CHG: N
      |                     ; P_COUT: N
      |                     ; P_CTMR: N
      |                     ; P_D1: A
      |                     ; P_R3: 2
      |                     ; P_R8: 2
      |                     ; P_RSHDN_PD: 2
      |                     ; P_U1: GND
      |                     ; Q2: 3(S)
      |                     ; Q3: 1(S1), 4(S2)
      |                     ; R1: 2(n)
      |                     ; R18: 2
      |                     ; R21: 2
      |                     ; R24: 2
      |                     ; R35: 2
      |                     ; R42: 2
      |                     ; R44: 2
      |                     ; R48: 2
      |                     ; U1: 8(CH7), 9(DGND), 14(AGND)
      |                     ; U2: 2(GND), 3(REF2), 4(RESERVED_GND)
      |                     ; U3: 2(GND), 3(REF2), 4(RESERVED_GND)
      |                     ; U4: 3(GND)
      |                     ; U5: 3(GND)
      |                     ; U6: 3(GND)
      |                     ; U7: 3(GND), 8(GND), 13(GND), 18(GND), 23(GND), 28(GND), 33(AGND), 38(GND)
      |                     ; U9: 4(VEE)
      |                     ; U10: 1(GNDP), 2(GNDP), 5(GNDP), 8(GNDP), 9(GNDP), 10(GNDP), 11(GNDP), 12(GNDP), 13(GNDP), 14(GNDP), 15(GNDP), 16(GNDP), 17(GNDP), 18(GNDP)
      |                     ; U11: 2(GND)
      |                     ; U12: 2(GND)
      | 接続部品数　　　　　; 72部品（部品番号で集計。同一ネット全体）
      | 接続端子数　　　　　; 99端子（423端子の部品対応表で集計。ラベル・境界ポートの重複は含めない）
      | この場所の端子数　　; 1端子／1部品（同名ラベルによる接続を除く）
      | 同階層同名ラベル数　; 75個（このラベル自身を含む）
      | 全階層の接続ラベル　; 87個（実際に同じノードへつながるラベル。名前が違う別名も含む）
      | 接続ルール　　　　　; 同じ階層の同じラベル名を仮想配線として結ぶ。別のSubsystem内とは名前だけでつながらず、明示的なConnection Portと配線をたどる。色は用途の表示であり接続を決めない。
      | 確認の範囲　　　　　; 現在の保存回路の端子・配線から求めた静的接続。抵抗やICの内部を導線として短絡せずに集計した。説明の更新は動作シミュレーション、タイミング、実部品の性能・実機動作を保証するものではない。
      | 記録の基準　　　　　; measurement_label_layout_20261022_r01/after_layout_graph.json。部品対応表は端子名の対応付けにのみ使用。
      | 
      | 【この説明欄の略語・記号】
      | 用語1　　　　　　　 ; DC：Direct Current（直流）。ここでは直流電源または直流成分。DCバイアスはコンデンサに重なる直流電圧を指す。
      | 用語2　　　　　　　 ; DC/DC：DC-to-DC Converter（直流電圧変換器）。直流入力を別の直流電圧へ変換する電源回路。絶縁の有無は個々の部品説明で確認する。
      | 用語3　　　　　　　 ; ADC：Analog-to-Digital Converter（アナログ・デジタル変換器）。測定電圧をデジタル値へ変換する回路。電流や温度も、センサーで電圧へ変換した後に読み取る。
      | 用語4　　　　　　　 ; IC：Integrated Circuit（集積回路）。複数の電子素子と機能を小さな半導体チップに集積した部品。
      | 用語5　　　　　　　 ; CH：Channel（測定チャネル）。CH0〜CH7はADCの入力番号であり、同時測定を意味しない。
      | 用語6　　　　　　　 ; MOSFET：Metal-Oxide-Semiconductor Field-Effect Transistor（金属・酸化膜・半導体構造の電界効果トランジスタ）。ゲートとソースの電圧でドレインとソースの導通を制御する素子。N-MOSはNチャネル型を表す。
      | 用語7　　　　　　　 ; LiFePO4：Lithium Iron Phosphate（リン酸鉄リチウム）。電池の正極材料を示す化学式。英語の頭文字を並べた略語ではない。
      | 用語8　　　　　　　 ; GND：Ground（回路の基準電位・電流帰路）。この図の共通基準。保護接地や大地への接続を意味するとは限らない。
      | 用語9　　　　　　　 ; AGND：Analog Ground（アナログ回路の基準端子）。アナログ部分の電流帰路。現図では共通GNDへ接続されるが、実装時の電流経路への配慮は別途必要。
      | 用語10　　　　　　　; DGND：Digital Ground（デジタル回路の基準端子）。デジタル部分の電流帰路。現図では共通GNDへ接続される。
      | 用語11　　　　　　　; VREF/REF：基準電圧を表す端子名。REFはReference（基準）の意味。ADCの変換尺度や電流アンプの出力基準に使う。REF1/REF2の接続電位は個別に確認する。
      | 用語12　　　　　　　; VCC/VDD/VEE/VS：ICの電源端子名。文字の歴史的な由来を現在の接続機能へ当てはめない。現回路のVEEはU8/U10では浮動基準SW、U9ではGND。各電圧・基準は端子と接続を参照する。
      | 用語13　　　　　　　; GNDP：U10の一次側電源の基準端子。絶縁電源の入力側GND。二次側基準VEE=SWと直接同一の導体ではない。
      | 用語14　　　　　　　; SW：Switching Node（スイッチング点）。主電力段の上下MOSFETとL1がつながる、電圧が高速に切り替わる点。GNDとは別電位。
  GND_Label_065 : ConnectionLabel  Description=|  Label=GND
      | この回路での名前　　; GND
      | 種別　　　　　　　　; ConnectionLabel
      | この回路での役割　　; 電池BT1の負極、太陽電池列の負極、制御・測定・保護回路のGNDを結ぶ共通の帰路。高側駆動の浮動帰路SWとは別のノード。
      | 共通帰路の代表接続　; BT1（充電先の蓄電池／51.2V 100Ah LiFePO4）: -
      |                     ; PV1（直列太陽電池列の負極側パネル／400W panel 1/2）: -
      |                     ; U7（RP2040搭載Pico W／SC0918）: 3(GND), 8(GND), 13(GND), 18(GND), 23(GND), 28(GND), 33(AGND), 38(GND)
      |                     ; U1（外付けADC／MCP3208-CI/SL）: 8(CH7), 9(DGND), 14(AGND)
      |                     ; P_U1（保護MOSFETを制御する保護IC／LTC4364IMS-1#PBF）: GND
      |                     ; Q2（同期整流降圧回路の下側スイッチ／TK9R6E15Q5,S1X）: 3(S)
      |                     ; U9（低側の光ゲートドライバ／ACPL-P346-560E）: 4(VEE)
      |                     ; U10（高側ゲート用の浮動電源を作る絶縁DC/DC／UCC14131QDWNRQ1）: 1(GNDP), 2(GNDP), 5(GNDP), 8(GNDP), 9(GNDP), 10(GNDP), 11(GNDP), 12(GNDP), 13(GNDP), 14(GNDP), 15(GNDP), 16(GNDP), 17(GNDP), 18(GNDP)
      | この場所の直接接続　; U1（外付けADC／MCP3208-CI/SL）: 14(AGND)
      | 直接接続の範囲　　　; このラベルから実際の線・分岐・明示的な境界端子だけを追った接続。同名ラベルによる離れた場所への接続はこの欄に含めない。
      | 同一ネット全端子　　; BT1: -
      |                     ; C1: 2(n)
      |                     ; C2: 2(n)
      |                     ; C3: 2(n)
      |                     ; C4: 2(n)
      |                     ; C7: 2(n)
      |                     ; C8: 2(n)
      |                     ; C9: 2(n)
      |                     ; C10: 2(n)
      |                     ; C13: 2(n)
      |                     ; C14: 2(n)
      |                     ; C15: 2(n)
      |                     ; C16: 2(n)
      |                     ; C17: 2
      |                     ; C18: 2
      |                     ; C19: 2
      |                     ; C20: 2
      |                     ; C21: 2
      |                     ; C22: 2
      |                     ; C23: 2
      |                     ; C24: 2
      |                     ; C25: 2
      |                     ; C26: 2
      |                     ; C27: 2
      |                     ; C28: 2
      |                     ; C29: 2
      |                     ; C30: 2
      |                     ; C31: 2
      |                     ; C33: 2
      |                     ; C34: 2
      |                     ; C35: 2
      |                     ; C36: 2
      |                     ; C40: 2
      |                     ; C41: 2
      |                     ; C42: 2
      |                     ; C43: 2
      |                     ; C44: 2
      |                     ; C45: 2
      |                     ; C46: 2
      |                     ; C47: 2
      |                     ; C48: 2
      |                     ; D2: 2(A)
      |                     ; PV1: -
      |                     ; P_CHG: N
      |                     ; P_COUT: N
      |                     ; P_CTMR: N
      |                     ; P_D1: A
      |                     ; P_R3: 2
      |                     ; P_R8: 2
      |                     ; P_RSHDN_PD: 2
      |                     ; P_U1: GND
      |                     ; Q2: 3(S)
      |                     ; Q3: 1(S1), 4(S2)
      |                     ; R1: 2(n)
      |                     ; R18: 2
      |                     ; R21: 2
      |                     ; R24: 2
      |                     ; R35: 2
      |                     ; R42: 2
      |                     ; R44: 2
      |                     ; R48: 2
      |                     ; U1: 8(CH7), 9(DGND), 14(AGND)
      |                     ; U2: 2(GND), 3(REF2), 4(RESERVED_GND)
      |                     ; U3: 2(GND), 3(REF2), 4(RESERVED_GND)
      |                     ; U4: 3(GND)
      |                     ; U5: 3(GND)
      |                     ; U6: 3(GND)
      |                     ; U7: 3(GND), 8(GND), 13(GND), 18(GND), 23(GND), 28(GND), 33(AGND), 38(GND)
      |                     ; U9: 4(VEE)
      |                     ; U10: 1(GNDP), 2(GNDP), 5(GNDP), 8(GNDP), 9(GNDP), 10(GNDP), 11(GNDP), 12(GNDP), 13(GNDP), 14(GNDP), 15(GNDP), 16(GNDP), 17(GNDP), 18(GNDP)
      |                     ; U11: 2(GND)
      |                     ; U12: 2(GND)
      | 接続部品数　　　　　; 72部品（部品番号で集計。同一ネット全体）
      | 接続端子数　　　　　; 99端子（423端子の部品対応表で集計。ラベル・境界ポートの重複は含めない）
      | この場所の端子数　　; 1端子／1部品（同名ラベルによる接続を除く）
      | 同階層同名ラベル数　; 75個（このラベル自身を含む）
      | 全階層の接続ラベル　; 87個（実際に同じノードへつながるラベル。名前が違う別名も含む）
      | 接続ルール　　　　　; 同じ階層の同じラベル名を仮想配線として結ぶ。別のSubsystem内とは名前だけでつながらず、明示的なConnection Portと配線をたどる。色は用途の表示であり接続を決めない。
      | 確認の範囲　　　　　; 現在の保存回路の端子・配線から求めた静的接続。抵抗やICの内部を導線として短絡せずに集計した。説明の更新は動作シミュレーション、タイミング、実部品の性能・実機動作を保証するものではない。
      | 記録の基準　　　　　; measurement_label_layout_20261022_r01/after_layout_graph.json。部品対応表は端子名の対応付けにのみ使用。
      | 
      | 【この説明欄の略語・記号】
      | 用語1　　　　　　　 ; DC：Direct Current（直流）。ここでは直流電源または直流成分。DCバイアスはコンデンサに重なる直流電圧を指す。
      | 用語2　　　　　　　 ; DC/DC：DC-to-DC Converter（直流電圧変換器）。直流入力を別の直流電圧へ変換する電源回路。絶縁の有無は個々の部品説明で確認する。
      | 用語3　　　　　　　 ; ADC：Analog-to-Digital Converter（アナログ・デジタル変換器）。測定電圧をデジタル値へ変換する回路。電流や温度も、センサーで電圧へ変換した後に読み取る。
      | 用語4　　　　　　　 ; IC：Integrated Circuit（集積回路）。複数の電子素子と機能を小さな半導体チップに集積した部品。
      | 用語5　　　　　　　 ; CH：Channel（測定チャネル）。CH0〜CH7はADCの入力番号であり、同時測定を意味しない。
      | 用語6　　　　　　　 ; MOSFET：Metal-Oxide-Semiconductor Field-Effect Transistor（金属・酸化膜・半導体構造の電界効果トランジスタ）。ゲートとソースの電圧でドレインとソースの導通を制御する素子。N-MOSはNチャネル型を表す。
      | 用語7　　　　　　　 ; LiFePO4：Lithium Iron Phosphate（リン酸鉄リチウム）。電池の正極材料を示す化学式。英語の頭文字を並べた略語ではない。
      | 用語8　　　　　　　 ; GND：Ground（回路の基準電位・電流帰路）。この図の共通基準。保護接地や大地への接続を意味するとは限らない。
      | 用語9　　　　　　　 ; AGND：Analog Ground（アナログ回路の基準端子）。アナログ部分の電流帰路。現図では共通GNDへ接続されるが、実装時の電流経路への配慮は別途必要。
      | 用語10　　　　　　　; DGND：Digital Ground（デジタル回路の基準端子）。デジタル部分の電流帰路。現図では共通GNDへ接続される。
      | 用語11　　　　　　　; VREF/REF：基準電圧を表す端子名。REFはReference（基準）の意味。ADCの変換尺度や電流アンプの出力基準に使う。REF1/REF2の接続電位は個別に確認する。
      | 用語12　　　　　　　; VCC/VDD/VEE/VS：ICの電源端子名。文字の歴史的な由来を現在の接続機能へ当てはめない。現回路のVEEはU8/U10では浮動基準SW、U9ではGND。各電圧・基準は端子と接続を参照する。
      | 用語13　　　　　　　; GNDP：U10の一次側電源の基準端子。絶縁電源の入力側GND。二次側基準VEE=SWと直接同一の導体ではない。
      | 用語14　　　　　　　; SW：Switching Node（スイッチング点）。主電力段の上下MOSFETとL1がつながる、電圧が高速に切り替わる点。GNDとは別電位。
  GND_Label_069 : ConnectionLabel  Description=|  Label=GND
      | この回路での名前　　; GND
      | 種別　　　　　　　　; ConnectionLabel
      | この回路での役割　　; 電池BT1の負極、太陽電池列の負極、制御・測定・保護回路のGNDを結ぶ共通の帰路。高側駆動の浮動帰路SWとは別のノード。
      | 共通帰路の代表接続　; BT1（充電先の蓄電池／51.2V 100Ah LiFePO4）: -
      |                     ; PV1（直列太陽電池列の負極側パネル／400W panel 1/2）: -
      |                     ; U7（RP2040搭載Pico W／SC0918）: 3(GND), 8(GND), 13(GND), 18(GND), 23(GND), 28(GND), 33(AGND), 38(GND)
      |                     ; U1（外付けADC／MCP3208-CI/SL）: 8(CH7), 9(DGND), 14(AGND)
      |                     ; P_U1（保護MOSFETを制御する保護IC／LTC4364IMS-1#PBF）: GND
      |                     ; Q2（同期整流降圧回路の下側スイッチ／TK9R6E15Q5,S1X）: 3(S)
      |                     ; U9（低側の光ゲートドライバ／ACPL-P346-560E）: 4(VEE)
      |                     ; U10（高側ゲート用の浮動電源を作る絶縁DC/DC／UCC14131QDWNRQ1）: 1(GNDP), 2(GNDP), 5(GNDP), 8(GNDP), 9(GNDP), 10(GNDP), 11(GNDP), 12(GNDP), 13(GNDP), 14(GNDP), 15(GNDP), 16(GNDP), 17(GNDP), 18(GNDP)
      | この場所の直接接続　; U10（高側ゲート用の浮動電源を作る絶縁DC/DC／UCC14131QDWNRQ1）: 1(GNDP), 2(GNDP), 5(GNDP), 8(GNDP), 9(GNDP), 10(GNDP), 11(GNDP), 12(GNDP), 13(GNDP), 14(GNDP), 15(GNDP), 16(GNDP), 17(GNDP), 18(GNDP)
      | 直接接続の範囲　　　; このラベルから実際の線・分岐・明示的な境界端子だけを追った接続。同名ラベルによる離れた場所への接続はこの欄に含めない。
      | 同一ネット全端子　　; BT1: -
      |                     ; C1: 2(n)
      |                     ; C2: 2(n)
      |                     ; C3: 2(n)
      |                     ; C4: 2(n)
      |                     ; C7: 2(n)
      |                     ; C8: 2(n)
      |                     ; C9: 2(n)
      |                     ; C10: 2(n)
      |                     ; C13: 2(n)
      |                     ; C14: 2(n)
      |                     ; C15: 2(n)
      |                     ; C16: 2(n)
      |                     ; C17: 2
      |                     ; C18: 2
      |                     ; C19: 2
      |                     ; C20: 2
      |                     ; C21: 2
      |                     ; C22: 2
      |                     ; C23: 2
      |                     ; C24: 2
      |                     ; C25: 2
      |                     ; C26: 2
      |                     ; C27: 2
      |                     ; C28: 2
      |                     ; C29: 2
      |                     ; C30: 2
      |                     ; C31: 2
      |                     ; C33: 2
      |                     ; C34: 2
      |                     ; C35: 2
      |                     ; C36: 2
      |                     ; C40: 2
      |                     ; C41: 2
      |                     ; C42: 2
      |                     ; C43: 2
      |                     ; C44: 2
      |                     ; C45: 2
      |                     ; C46: 2
      |                     ; C47: 2
      |                     ; C48: 2
      |                     ; D2: 2(A)
      |                     ; PV1: -
      |                     ; P_CHG: N
      |                     ; P_COUT: N
      |                     ; P_CTMR: N
      |                     ; P_D1: A
      |                     ; P_R3: 2
      |                     ; P_R8: 2
      |                     ; P_RSHDN_PD: 2
      |                     ; P_U1: GND
      |                     ; Q2: 3(S)
      |                     ; Q3: 1(S1), 4(S2)
      |                     ; R1: 2(n)
      |                     ; R18: 2
      |                     ; R21: 2
      |                     ; R24: 2
      |                     ; R35: 2
      |                     ; R42: 2
      |                     ; R44: 2
      |                     ; R48: 2
      |                     ; U1: 8(CH7), 9(DGND), 14(AGND)
      |                     ; U2: 2(GND), 3(REF2), 4(RESERVED_GND)
      |                     ; U3: 2(GND), 3(REF2), 4(RESERVED_GND)
      |                     ; U4: 3(GND)
      |                     ; U5: 3(GND)
      |                     ; U6: 3(GND)
      |                     ; U7: 3(GND), 8(GND), 13(GND), 18(GND), 23(GND), 28(GND), 33(AGND), 38(GND)
      |                     ; U9: 4(VEE)
      |                     ; U10: 1(GNDP), 2(GNDP), 5(GNDP), 8(GNDP), 9(GNDP), 10(GNDP), 11(GNDP), 12(GNDP), 13(GNDP), 14(GNDP), 15(GNDP), 16(GNDP), 17(GNDP), 18(GNDP)
      |                     ; U11: 2(GND)
      |                     ; U12: 2(GND)
      | 接続部品数　　　　　; 72部品（部品番号で集計。同一ネット全体）
      | 接続端子数　　　　　; 99端子（423端子の部品対応表で集計。ラベル・境界ポートの重複は含めない）
      | この場所の端子数　　; 14端子／1部品（同名ラベルによる接続を除く）
      | 同階層同名ラベル数　; 75個（このラベル自身を含む）
      | 全階層の接続ラベル　; 87個（実際に同じノードへつながるラベル。名前が違う別名も含む）
      | 接続ルール　　　　　; 同じ階層の同じラベル名を仮想配線として結ぶ。別のSubsystem内とは名前だけでつながらず、明示的なConnection Portと配線をたどる。色は用途の表示であり接続を決めない。
      | 確認の範囲　　　　　; 現在の保存回路の端子・配線から求めた静的接続。抵抗やICの内部を導線として短絡せずに集計した。説明の更新は動作シミュレーション、タイミング、実部品の性能・実機動作を保証するものではない。
      | 記録の基準　　　　　; measurement_label_layout_20261022_r01/after_layout_graph.json。部品対応表は端子名の対応付けにのみ使用。
      | 
      | 【この説明欄の略語・記号】
      | 用語1　　　　　　　 ; DC：Direct Current（直流）。ここでは直流電源または直流成分。DCバイアスはコンデンサに重なる直流電圧を指す。
      | 用語2　　　　　　　 ; DC/DC：DC-to-DC Converter（直流電圧変換器）。直流入力を別の直流電圧へ変換する電源回路。絶縁の有無は個々の部品説明で確認する。
      | 用語3　　　　　　　 ; ADC：Analog-to-Digital Converter（アナログ・デジタル変換器）。測定電圧をデジタル値へ変換する回路。電流や温度も、センサーで電圧へ変換した後に読み取る。
      | 用語4　　　　　　　 ; IC：Integrated Circuit（集積回路）。複数の電子素子と機能を小さな半導体チップに集積した部品。
      | 用語5　　　　　　　 ; CH：Channel（測定チャネル）。CH0〜CH7はADCの入力番号であり、同時測定を意味しない。
      | 用語6　　　　　　　 ; MOSFET：Metal-Oxide-Semiconductor Field-Effect Transistor（金属・酸化膜・半導体構造の電界効果トランジスタ）。ゲートとソースの電圧でドレインとソースの導通を制御する素子。N-MOSはNチャネル型を表す。
      | 用語7　　　　　　　 ; LiFePO4：Lithium Iron Phosphate（リン酸鉄リチウム）。電池の正極材料を示す化学式。英語の頭文字を並べた略語ではない。
      | 用語8　　　　　　　 ; GND：Ground（回路の基準電位・電流帰路）。この図の共通基準。保護接地や大地への接続を意味するとは限らない。
      | 用語9　　　　　　　 ; AGND：Analog Ground（アナログ回路の基準端子）。アナログ部分の電流帰路。現図では共通GNDへ接続されるが、実装時の電流経路への配慮は別途必要。
      | 用語10　　　　　　　; DGND：Digital Ground（デジタル回路の基準端子）。デジタル部分の電流帰路。現図では共通GNDへ接続される。
      | 用語11　　　　　　　; VREF/REF：基準電圧を表す端子名。REFはReference（基準）の意味。ADCの変換尺度や電流アンプの出力基準に使う。REF1/REF2の接続電位は個別に確認する。
      | 用語12　　　　　　　; VCC/VDD/VEE/VS：ICの電源端子名。文字の歴史的な由来を現在の接続機能へ当てはめない。現回路のVEEはU8/U10では浮動基準SW、U9ではGND。各電圧・基準は端子と接続を参照する。
      | 用語13　　　　　　　; GNDP：U10の一次側電源の基準端子。絶縁電源の入力側GND。二次側基準VEE=SWと直接同一の導体ではない。
      | 用語14　　　　　　　; SW：Switching Node（スイッチング点）。主電力段の上下MOSFETとL1がつながる、電圧が高速に切り替わる点。GNDとは別電位。
  GND_Label_080 : ConnectionLabel  Description=|  Label=GND
      | この回路での名前　　; GND
      | 種別　　　　　　　　; ConnectionLabel
      | この回路での役割　　; 電池BT1の負極、太陽電池列の負極、制御・測定・保護回路のGNDを結ぶ共通の帰路。高側駆動の浮動帰路SWとは別のノード。
      | 共通帰路の代表接続　; BT1（充電先の蓄電池／51.2V 100Ah LiFePO4）: -
      |                     ; PV1（直列太陽電池列の負極側パネル／400W panel 1/2）: -
      |                     ; U7（RP2040搭載Pico W／SC0918）: 3(GND), 8(GND), 13(GND), 18(GND), 23(GND), 28(GND), 33(AGND), 38(GND)
      |                     ; U1（外付けADC／MCP3208-CI/SL）: 8(CH7), 9(DGND), 14(AGND)
      |                     ; P_U1（保護MOSFETを制御する保護IC／LTC4364IMS-1#PBF）: GND
      |                     ; Q2（同期整流降圧回路の下側スイッチ／TK9R6E15Q5,S1X）: 3(S)
      |                     ; U9（低側の光ゲートドライバ／ACPL-P346-560E）: 4(VEE)
      |                     ; U10（高側ゲート用の浮動電源を作る絶縁DC/DC／UCC14131QDWNRQ1）: 1(GNDP), 2(GNDP), 5(GNDP), 8(GNDP), 9(GNDP), 10(GNDP), 11(GNDP), 12(GNDP), 13(GNDP), 14(GNDP), 15(GNDP), 16(GNDP), 17(GNDP), 18(GNDP)
      | この場所の直接接続　; U11（バッテリー補助分岐から12Vを作る電源モジュール／TSR 1-48120WI）: 2(GND)
      | 直接接続の範囲　　　; このラベルから実際の線・分岐・明示的な境界端子だけを追った接続。同名ラベルによる離れた場所への接続はこの欄に含めない。
      | 同一ネット全端子　　; BT1: -
      |                     ; C1: 2(n)
      |                     ; C2: 2(n)
      |                     ; C3: 2(n)
      |                     ; C4: 2(n)
      |                     ; C7: 2(n)
      |                     ; C8: 2(n)
      |                     ; C9: 2(n)
      |                     ; C10: 2(n)
      |                     ; C13: 2(n)
      |                     ; C14: 2(n)
      |                     ; C15: 2(n)
      |                     ; C16: 2(n)
      |                     ; C17: 2
      |                     ; C18: 2
      |                     ; C19: 2
      |                     ; C20: 2
      |                     ; C21: 2
      |                     ; C22: 2
      |                     ; C23: 2
      |                     ; C24: 2
      |                     ; C25: 2
      |                     ; C26: 2
      |                     ; C27: 2
      |                     ; C28: 2
      |                     ; C29: 2
      |                     ; C30: 2
      |                     ; C31: 2
      |                     ; C33: 2
      |                     ; C34: 2
      |                     ; C35: 2
      |                     ; C36: 2
      |                     ; C40: 2
      |                     ; C41: 2
      |                     ; C42: 2
      |                     ; C43: 2
      |                     ; C44: 2
      |                     ; C45: 2
      |                     ; C46: 2
      |                     ; C47: 2
      |                     ; C48: 2
      |                     ; D2: 2(A)
      |                     ; PV1: -
      |                     ; P_CHG: N
      |                     ; P_COUT: N
      |                     ; P_CTMR: N
      |                     ; P_D1: A
      |                     ; P_R3: 2
      |                     ; P_R8: 2
      |                     ; P_RSHDN_PD: 2
      |                     ; P_U1: GND
      |                     ; Q2: 3(S)
      |                     ; Q3: 1(S1), 4(S2)
      |                     ; R1: 2(n)
      |                     ; R18: 2
      |                     ; R21: 2
      |                     ; R24: 2
      |                     ; R35: 2
      |                     ; R42: 2
      |                     ; R44: 2
      |                     ; R48: 2
      |                     ; U1: 8(CH7), 9(DGND), 14(AGND)
      |                     ; U2: 2(GND), 3(REF2), 4(RESERVED_GND)
      |                     ; U3: 2(GND), 3(REF2), 4(RESERVED_GND)
      |                     ; U4: 3(GND)
      |                     ; U5: 3(GND)
      |                     ; U6: 3(GND)
      |                     ; U7: 3(GND), 8(GND), 13(GND), 18(GND), 23(GND), 28(GND), 33(AGND), 38(GND)
      |                     ; U9: 4(VEE)
      |                     ; U10: 1(GNDP), 2(GNDP), 5(GNDP), 8(GNDP), 9(GNDP), 10(GNDP), 11(GNDP), 12(GNDP), 13(GNDP), 14(GNDP), 15(GNDP), 16(GNDP), 17(GNDP), 18(GNDP)
      |                     ; U11: 2(GND)
      |                     ; U12: 2(GND)
      | 接続部品数　　　　　; 72部品（部品番号で集計。同一ネット全体）
      | 接続端子数　　　　　; 99端子（423端子の部品対応表で集計。ラベル・境界ポートの重複は含めない）
      | この場所の端子数　　; 1端子／1部品（同名ラベルによる接続を除く）
      | 同階層同名ラベル数　; 75個（このラベル自身を含む）
      | 全階層の接続ラベル　; 87個（実際に同じノードへつながるラベル。名前が違う別名も含む）
      | 接続ルール　　　　　; 同じ階層の同じラベル名を仮想配線として結ぶ。別のSubsystem内とは名前だけでつながらず、明示的なConnection Portと配線をたどる。色は用途の表示であり接続を決めない。
      | 確認の範囲　　　　　; 現在の保存回路の端子・配線から求めた静的接続。抵抗やICの内部を導線として短絡せずに集計した。説明の更新は動作シミュレーション、タイミング、実部品の性能・実機動作を保証するものではない。
      | 記録の基準　　　　　; measurement_label_layout_20261022_r01/after_layout_graph.json。部品対応表は端子名の対応付けにのみ使用。
      | 
      | 【この説明欄の略語・記号】
      | 用語1　　　　　　　 ; DC：Direct Current（直流）。ここでは直流電源または直流成分。DCバイアスはコンデンサに重なる直流電圧を指す。
      | 用語2　　　　　　　 ; DC/DC：DC-to-DC Converter（直流電圧変換器）。直流入力を別の直流電圧へ変換する電源回路。絶縁の有無は個々の部品説明で確認する。
      | 用語3　　　　　　　 ; ADC：Analog-to-Digital Converter（アナログ・デジタル変換器）。測定電圧をデジタル値へ変換する回路。電流や温度も、センサーで電圧へ変換した後に読み取る。
      | 用語4　　　　　　　 ; IC：Integrated Circuit（集積回路）。複数の電子素子と機能を小さな半導体チップに集積した部品。
      | 用語5　　　　　　　 ; CH：Channel（測定チャネル）。CH0〜CH7はADCの入力番号であり、同時測定を意味しない。
      | 用語6　　　　　　　 ; MOSFET：Metal-Oxide-Semiconductor Field-Effect Transistor（金属・酸化膜・半導体構造の電界効果トランジスタ）。ゲートとソースの電圧でドレインとソースの導通を制御する素子。N-MOSはNチャネル型を表す。
      | 用語7　　　　　　　 ; LiFePO4：Lithium Iron Phosphate（リン酸鉄リチウム）。電池の正極材料を示す化学式。英語の頭文字を並べた略語ではない。
      | 用語8　　　　　　　 ; GND：Ground（回路の基準電位・電流帰路）。この図の共通基準。保護接地や大地への接続を意味するとは限らない。
      | 用語9　　　　　　　 ; AGND：Analog Ground（アナログ回路の基準端子）。アナログ部分の電流帰路。現図では共通GNDへ接続されるが、実装時の電流経路への配慮は別途必要。
      | 用語10　　　　　　　; DGND：Digital Ground（デジタル回路の基準端子）。デジタル部分の電流帰路。現図では共通GNDへ接続される。
      | 用語11　　　　　　　; VREF/REF：基準電圧を表す端子名。REFはReference（基準）の意味。ADCの変換尺度や電流アンプの出力基準に使う。REF1/REF2の接続電位は個別に確認する。
      | 用語12　　　　　　　; VCC/VDD/VEE/VS：ICの電源端子名。文字の歴史的な由来を現在の接続機能へ当てはめない。現回路のVEEはU8/U10では浮動基準SW、U9ではGND。各電圧・基準は端子と接続を参照する。
      | 用語13　　　　　　　; GNDP：U10の一次側電源の基準端子。絶縁電源の入力側GND。二次側基準VEE=SWと直接同一の導体ではない。
      | 用語14　　　　　　　; SW：Switching Node（スイッチング点）。主電力段の上下MOSFETとL1がつながる、電圧が高速に切り替わる点。GNDとは別電位。
  GND_Label_081 : ConnectionLabel  Description=|  Label=GND
      | この回路での名前　　; GND
      | 種別　　　　　　　　; ConnectionLabel
      | この回路での役割　　; 電池BT1の負極、太陽電池列の負極、制御・測定・保護回路のGNDを結ぶ共通の帰路。高側駆動の浮動帰路SWとは別のノード。
      | 共通帰路の代表接続　; BT1（充電先の蓄電池／51.2V 100Ah LiFePO4）: -
      |                     ; PV1（直列太陽電池列の負極側パネル／400W panel 1/2）: -
      |                     ; U7（RP2040搭載Pico W／SC0918）: 3(GND), 8(GND), 13(GND), 18(GND), 23(GND), 28(GND), 33(AGND), 38(GND)
      |                     ; U1（外付けADC／MCP3208-CI/SL）: 8(CH7), 9(DGND), 14(AGND)
      |                     ; P_U1（保護MOSFETを制御する保護IC／LTC4364IMS-1#PBF）: GND
      |                     ; Q2（同期整流降圧回路の下側スイッチ／TK9R6E15Q5,S1X）: 3(S)
      |                     ; U9（低側の光ゲートドライバ／ACPL-P346-560E）: 4(VEE)
      |                     ; U10（高側ゲート用の浮動電源を作る絶縁DC/DC／UCC14131QDWNRQ1）: 1(GNDP), 2(GNDP), 5(GNDP), 8(GNDP), 9(GNDP), 10(GNDP), 11(GNDP), 12(GNDP), 13(GNDP), 14(GNDP), 15(GNDP), 16(GNDP), 17(GNDP), 18(GNDP)
      | この場所の直接接続　; U12（12Vから5Vを作る電源モジュール／TSR 1-2450）: 2(GND)
      | 直接接続の範囲　　　; このラベルから実際の線・分岐・明示的な境界端子だけを追った接続。同名ラベルによる離れた場所への接続はこの欄に含めない。
      | 同一ネット全端子　　; BT1: -
      |                     ; C1: 2(n)
      |                     ; C2: 2(n)
      |                     ; C3: 2(n)
      |                     ; C4: 2(n)
      |                     ; C7: 2(n)
      |                     ; C8: 2(n)
      |                     ; C9: 2(n)
      |                     ; C10: 2(n)
      |                     ; C13: 2(n)
      |                     ; C14: 2(n)
      |                     ; C15: 2(n)
      |                     ; C16: 2(n)
      |                     ; C17: 2
      |                     ; C18: 2
      |                     ; C19: 2
      |                     ; C20: 2
      |                     ; C21: 2
      |                     ; C22: 2
      |                     ; C23: 2
      |                     ; C24: 2
      |                     ; C25: 2
      |                     ; C26: 2
      |                     ; C27: 2
      |                     ; C28: 2
      |                     ; C29: 2
      |                     ; C30: 2
      |                     ; C31: 2
      |                     ; C33: 2
      |                     ; C34: 2
      |                     ; C35: 2
      |                     ; C36: 2
      |                     ; C40: 2
      |                     ; C41: 2
      |                     ; C42: 2
      |                     ; C43: 2
      |                     ; C44: 2
      |                     ; C45: 2
      |                     ; C46: 2
      |                     ; C47: 2
      |                     ; C48: 2
      |                     ; D2: 2(A)
      |                     ; PV1: -
      |                     ; P_CHG: N
      |                     ; P_COUT: N
      |                     ; P_CTMR: N
      |                     ; P_D1: A
      |                     ; P_R3: 2
      |                     ; P_R8: 2
      |                     ; P_RSHDN_PD: 2
      |                     ; P_U1: GND
      |                     ; Q2: 3(S)
      |                     ; Q3: 1(S1), 4(S2)
      |                     ; R1: 2(n)
      |                     ; R18: 2
      |                     ; R21: 2
      |                     ; R24: 2
      |                     ; R35: 2
      |                     ; R42: 2
      |                     ; R44: 2
      |                     ; R48: 2
      |                     ; U1: 8(CH7), 9(DGND), 14(AGND)
      |                     ; U2: 2(GND), 3(REF2), 4(RESERVED_GND)
      |                     ; U3: 2(GND), 3(REF2), 4(RESERVED_GND)
      |                     ; U4: 3(GND)
      |                     ; U5: 3(GND)
      |                     ; U6: 3(GND)
      |                     ; U7: 3(GND), 8(GND), 13(GND), 18(GND), 23(GND), 28(GND), 33(AGND), 38(GND)
      |                     ; U9: 4(VEE)
      |                     ; U10: 1(GNDP), 2(GNDP), 5(GNDP), 8(GNDP), 9(GNDP), 10(GNDP), 11(GNDP), 12(GNDP), 13(GNDP), 14(GNDP), 15(GNDP), 16(GNDP), 17(GNDP), 18(GNDP)
      |                     ; U11: 2(GND)
      |                     ; U12: 2(GND)
      | 接続部品数　　　　　; 72部品（部品番号で集計。同一ネット全体）
      | 接続端子数　　　　　; 99端子（423端子の部品対応表で集計。ラベル・境界ポートの重複は含めない）
      | この場所の端子数　　; 1端子／1部品（同名ラベルによる接続を除く）
      | 同階層同名ラベル数　; 75個（このラベル自身を含む）
      | 全階層の接続ラベル　; 87個（実際に同じノードへつながるラベル。名前が違う別名も含む）
      | 接続ルール　　　　　; 同じ階層の同じラベル名を仮想配線として結ぶ。別のSubsystem内とは名前だけでつながらず、明示的なConnection Portと配線をたどる。色は用途の表示であり接続を決めない。
      | 確認の範囲　　　　　; 現在の保存回路の端子・配線から求めた静的接続。抵抗やICの内部を導線として短絡せずに集計した。説明の更新は動作シミュレーション、タイミング、実部品の性能・実機動作を保証するものではない。
      | 記録の基準　　　　　; measurement_label_layout_20261022_r01/after_layout_graph.json。部品対応表は端子名の対応付けにのみ使用。
      | 
      | 【この説明欄の略語・記号】
      | 用語1　　　　　　　 ; DC：Direct Current（直流）。ここでは直流電源または直流成分。DCバイアスはコンデンサに重なる直流電圧を指す。
      | 用語2　　　　　　　 ; DC/DC：DC-to-DC Converter（直流電圧変換器）。直流入力を別の直流電圧へ変換する電源回路。絶縁の有無は個々の部品説明で確認する。
      | 用語3　　　　　　　 ; ADC：Analog-to-Digital Converter（アナログ・デジタル変換器）。測定電圧をデジタル値へ変換する回路。電流や温度も、センサーで電圧へ変換した後に読み取る。
      | 用語4　　　　　　　 ; IC：Integrated Circuit（集積回路）。複数の電子素子と機能を小さな半導体チップに集積した部品。
      | 用語5　　　　　　　 ; CH：Channel（測定チャネル）。CH0〜CH7はADCの入力番号であり、同時測定を意味しない。
      | 用語6　　　　　　　 ; MOSFET：Metal-Oxide-Semiconductor Field-Effect Transistor（金属・酸化膜・半導体構造の電界効果トランジスタ）。ゲートとソースの電圧でドレインとソースの導通を制御する素子。N-MOSはNチャネル型を表す。
      | 用語7　　　　　　　 ; LiFePO4：Lithium Iron Phosphate（リン酸鉄リチウム）。電池の正極材料を示す化学式。英語の頭文字を並べた略語ではない。
      | 用語8　　　　　　　 ; GND：Ground（回路の基準電位・電流帰路）。この図の共通基準。保護接地や大地への接続を意味するとは限らない。
      | 用語9　　　　　　　 ; AGND：Analog Ground（アナログ回路の基準端子）。アナログ部分の電流帰路。現図では共通GNDへ接続されるが、実装時の電流経路への配慮は別途必要。
      | 用語10　　　　　　　; DGND：Digital Ground（デジタル回路の基準端子）。デジタル部分の電流帰路。現図では共通GNDへ接続される。
      | 用語11　　　　　　　; VREF/REF：基準電圧を表す端子名。REFはReference（基準）の意味。ADCの変換尺度や電流アンプの出力基準に使う。REF1/REF2の接続電位は個別に確認する。
      | 用語12　　　　　　　; VCC/VDD/VEE/VS：ICの電源端子名。文字の歴史的な由来を現在の接続機能へ当てはめない。現回路のVEEはU8/U10では浮動基準SW、U9ではGND。各電圧・基準は端子と接続を参照する。
      | 用語13　　　　　　　; GNDP：U10の一次側電源の基準端子。絶縁電源の入力側GND。二次側基準VEE=SWと直接同一の導体ではない。
      | 用語14　　　　　　　; SW：Switching Node（スイッチング点）。主電力段の上下MOSFETとL1がつながる、電圧が高速に切り替わる点。GNDとは別電位。
  GND_Label_085 : ConnectionLabel  Description=|  Label=GND
      | この回路での名前　　; GND
      | 種別　　　　　　　　; ConnectionLabel
      | この回路での役割　　; 電池BT1の負極、太陽電池列の負極、制御・測定・保護回路のGNDを結ぶ共通の帰路。高側駆動の浮動帰路SWとは別のノード。
      | 共通帰路の代表接続　; BT1（充電先の蓄電池／51.2V 100Ah LiFePO4）: -
      |                     ; PV1（直列太陽電池列の負極側パネル／400W panel 1/2）: -
      |                     ; U7（RP2040搭載Pico W／SC0918）: 3(GND), 8(GND), 13(GND), 18(GND), 23(GND), 28(GND), 33(AGND), 38(GND)
      |                     ; U1（外付けADC／MCP3208-CI/SL）: 8(CH7), 9(DGND), 14(AGND)
      |                     ; P_U1（保護MOSFETを制御する保護IC／LTC4364IMS-1#PBF）: GND
      |                     ; Q2（同期整流降圧回路の下側スイッチ／TK9R6E15Q5,S1X）: 3(S)
      |                     ; U9（低側の光ゲートドライバ／ACPL-P346-560E）: 4(VEE)
      |                     ; U10（高側ゲート用の浮動電源を作る絶縁DC/DC／UCC14131QDWNRQ1）: 1(GNDP), 2(GNDP), 5(GNDP), 8(GNDP), 9(GNDP), 10(GNDP), 11(GNDP), 12(GNDP), 13(GNDP), 14(GNDP), 15(GNDP), 16(GNDP), 17(GNDP), 18(GNDP)
      | この場所の直接接続　; U3（L1直後の出力電流の検出アンプ／INA241A3IDDFR）: 2(GND)
      | 直接接続の範囲　　　; このラベルから実際の線・分岐・明示的な境界端子だけを追った接続。同名ラベルによる離れた場所への接続はこの欄に含めない。
      | 同一ネット全端子　　; BT1: -
      |                     ; C1: 2(n)
      |                     ; C2: 2(n)
      |                     ; C3: 2(n)
      |                     ; C4: 2(n)
      |                     ; C7: 2(n)
      |                     ; C8: 2(n)
      |                     ; C9: 2(n)
      |                     ; C10: 2(n)
      |                     ; C13: 2(n)
      |                     ; C14: 2(n)
      |                     ; C15: 2(n)
      |                     ; C16: 2(n)
      |                     ; C17: 2
      |                     ; C18: 2
      |                     ; C19: 2
      |                     ; C20: 2
      |                     ; C21: 2
      |                     ; C22: 2
      |                     ; C23: 2
      |                     ; C24: 2
      |                     ; C25: 2
      |                     ; C26: 2
      |                     ; C27: 2
      |                     ; C28: 2
      |                     ; C29: 2
      |                     ; C30: 2
      |                     ; C31: 2
      |                     ; C33: 2
      |                     ; C34: 2
      |                     ; C35: 2
      |                     ; C36: 2
      |                     ; C40: 2
      |                     ; C41: 2
      |                     ; C42: 2
      |                     ; C43: 2
      |                     ; C44: 2
      |                     ; C45: 2
      |                     ; C46: 2
      |                     ; C47: 2
      |                     ; C48: 2
      |                     ; D2: 2(A)
      |                     ; PV1: -
      |                     ; P_CHG: N
      |                     ; P_COUT: N
      |                     ; P_CTMR: N
      |                     ; P_D1: A
      |                     ; P_R3: 2
      |                     ; P_R8: 2
      |                     ; P_RSHDN_PD: 2
      |                     ; P_U1: GND
      |                     ; Q2: 3(S)
      |                     ; Q3: 1(S1), 4(S2)
      |                     ; R1: 2(n)
      |                     ; R18: 2
      |                     ; R21: 2
      |                     ; R24: 2
      |                     ; R35: 2
      |                     ; R42: 2
      |                     ; R44: 2
      |                     ; R48: 2
      |                     ; U1: 8(CH7), 9(DGND), 14(AGND)
      |                     ; U2: 2(GND), 3(REF2), 4(RESERVED_GND)
      |                     ; U3: 2(GND), 3(REF2), 4(RESERVED_GND)
      |                     ; U4: 3(GND)
      |                     ; U5: 3(GND)
      |                     ; U6: 3(GND)
      |                     ; U7: 3(GND), 8(GND), 13(GND), 18(GND), 23(GND), 28(GND), 33(AGND), 38(GND)
      |                     ; U9: 4(VEE)
      |                     ; U10: 1(GNDP), 2(GNDP), 5(GNDP), 8(GNDP), 9(GNDP), 10(GNDP), 11(GNDP), 12(GNDP), 13(GNDP), 14(GNDP), 15(GNDP), 16(GNDP), 17(GNDP), 18(GNDP)
      |                     ; U11: 2(GND)
      |                     ; U12: 2(GND)
      | 接続部品数　　　　　; 72部品（部品番号で集計。同一ネット全体）
      | 接続端子数　　　　　; 99端子（423端子の部品対応表で集計。ラベル・境界ポートの重複は含めない）
      | この場所の端子数　　; 1端子／1部品（同名ラベルによる接続を除く）
      | 同階層同名ラベル数　; 75個（このラベル自身を含む）
      | 全階層の接続ラベル　; 87個（実際に同じノードへつながるラベル。名前が違う別名も含む）
      | 接続ルール　　　　　; 同じ階層の同じラベル名を仮想配線として結ぶ。別のSubsystem内とは名前だけでつながらず、明示的なConnection Portと配線をたどる。色は用途の表示であり接続を決めない。
      | 確認の範囲　　　　　; 現在の保存回路の端子・配線から求めた静的接続。抵抗やICの内部を導線として短絡せずに集計した。説明の更新は動作シミュレーション、タイミング、実部品の性能・実機動作を保証するものではない。
      | 記録の基準　　　　　; measurement_label_layout_20261022_r01/after_layout_graph.json。部品対応表は端子名の対応付けにのみ使用。
      | 
      | 【この説明欄の略語・記号】
      | 用語1　　　　　　　 ; DC：Direct Current（直流）。ここでは直流電源または直流成分。DCバイアスはコンデンサに重なる直流電圧を指す。
      | 用語2　　　　　　　 ; DC/DC：DC-to-DC Converter（直流電圧変換器）。直流入力を別の直流電圧へ変換する電源回路。絶縁の有無は個々の部品説明で確認する。
      | 用語3　　　　　　　 ; ADC：Analog-to-Digital Converter（アナログ・デジタル変換器）。測定電圧をデジタル値へ変換する回路。電流や温度も、センサーで電圧へ変換した後に読み取る。
      | 用語4　　　　　　　 ; IC：Integrated Circuit（集積回路）。複数の電子素子と機能を小さな半導体チップに集積した部品。
      | 用語5　　　　　　　 ; CH：Channel（測定チャネル）。CH0〜CH7はADCの入力番号であり、同時測定を意味しない。
      | 用語6　　　　　　　 ; MOSFET：Metal-Oxide-Semiconductor Field-Effect Transistor（金属・酸化膜・半導体構造の電界効果トランジスタ）。ゲートとソースの電圧でドレインとソースの導通を制御する素子。N-MOSはNチャネル型を表す。
      | 用語7　　　　　　　 ; LiFePO4：Lithium Iron Phosphate（リン酸鉄リチウム）。電池の正極材料を示す化学式。英語の頭文字を並べた略語ではない。
      | 用語8　　　　　　　 ; GND：Ground（回路の基準電位・電流帰路）。この図の共通基準。保護接地や大地への接続を意味するとは限らない。
      | 用語9　　　　　　　 ; AGND：Analog Ground（アナログ回路の基準端子）。アナログ部分の電流帰路。現図では共通GNDへ接続されるが、実装時の電流経路への配慮は別途必要。
      | 用語10　　　　　　　; DGND：Digital Ground（デジタル回路の基準端子）。デジタル部分の電流帰路。現図では共通GNDへ接続される。
      | 用語11　　　　　　　; VREF/REF：基準電圧を表す端子名。REFはReference（基準）の意味。ADCの変換尺度や電流アンプの出力基準に使う。REF1/REF2の接続電位は個別に確認する。
      | 用語12　　　　　　　; VCC/VDD/VEE/VS：ICの電源端子名。文字の歴史的な由来を現在の接続機能へ当てはめない。現回路のVEEはU8/U10では浮動基準SW、U9ではGND。各電圧・基準は端子と接続を参照する。
      | 用語13　　　　　　　; GNDP：U10の一次側電源の基準端子。絶縁電源の入力側GND。二次側基準VEE=SWと直接同一の導体ではない。
      | 用語14　　　　　　　; SW：Switching Node（スイッチング点）。主電力段の上下MOSFETとL1がつながる、電圧が高速に切り替わる点。GNDとは別電位。
  GND_Label_086 : ConnectionLabel  Description=|  Label=GND
      | この回路での名前　　; GND
      | 種別　　　　　　　　; ConnectionLabel
      | この回路での役割　　; 電池BT1の負極、太陽電池列の負極、制御・測定・保護回路のGNDを結ぶ共通の帰路。高側駆動の浮動帰路SWとは別のノード。
      | 共通帰路の代表接続　; BT1（充電先の蓄電池／51.2V 100Ah LiFePO4）: -
      |                     ; PV1（直列太陽電池列の負極側パネル／400W panel 1/2）: -
      |                     ; U7（RP2040搭載Pico W／SC0918）: 3(GND), 8(GND), 13(GND), 18(GND), 23(GND), 28(GND), 33(AGND), 38(GND)
      |                     ; U1（外付けADC／MCP3208-CI/SL）: 8(CH7), 9(DGND), 14(AGND)
      |                     ; P_U1（保護MOSFETを制御する保護IC／LTC4364IMS-1#PBF）: GND
      |                     ; Q2（同期整流降圧回路の下側スイッチ／TK9R6E15Q5,S1X）: 3(S)
      |                     ; U9（低側の光ゲートドライバ／ACPL-P346-560E）: 4(VEE)
      |                     ; U10（高側ゲート用の浮動電源を作る絶縁DC/DC／UCC14131QDWNRQ1）: 1(GNDP), 2(GNDP), 5(GNDP), 8(GNDP), 9(GNDP), 10(GNDP), 11(GNDP), 12(GNDP), 13(GNDP), 14(GNDP), 15(GNDP), 16(GNDP), 17(GNDP), 18(GNDP)
      | この場所の直接接続　; U3（L1直後の出力電流の検出アンプ／INA241A3IDDFR）: 3(REF2)
      | 直接接続の範囲　　　; このラベルから実際の線・分岐・明示的な境界端子だけを追った接続。同名ラベルによる離れた場所への接続はこの欄に含めない。
      | 同一ネット全端子　　; BT1: -
      |                     ; C1: 2(n)
      |                     ; C2: 2(n)
      |                     ; C3: 2(n)
      |                     ; C4: 2(n)
      |                     ; C7: 2(n)
      |                     ; C8: 2(n)
      |                     ; C9: 2(n)
      |                     ; C10: 2(n)
      |                     ; C13: 2(n)
      |                     ; C14: 2(n)
      |                     ; C15: 2(n)
      |                     ; C16: 2(n)
      |                     ; C17: 2
      |                     ; C18: 2
      |                     ; C19: 2
      |                     ; C20: 2
      |                     ; C21: 2
      |                     ; C22: 2
      |                     ; C23: 2
      |                     ; C24: 2
      |                     ; C25: 2
      |                     ; C26: 2
      |                     ; C27: 2
      |                     ; C28: 2
      |                     ; C29: 2
      |                     ; C30: 2
      |                     ; C31: 2
      |                     ; C33: 2
      |                     ; C34: 2
      |                     ; C35: 2
      |                     ; C36: 2
      |                     ; C40: 2
      |                     ; C41: 2
      |                     ; C42: 2
      |                     ; C43: 2
      |                     ; C44: 2
      |                     ; C45: 2
      |                     ; C46: 2
      |                     ; C47: 2
      |                     ; C48: 2
      |                     ; D2: 2(A)
      |                     ; PV1: -
      |                     ; P_CHG: N
      |                     ; P_COUT: N
      |                     ; P_CTMR: N
      |                     ; P_D1: A
      |                     ; P_R3: 2
      |                     ; P_R8: 2
      |                     ; P_RSHDN_PD: 2
      |                     ; P_U1: GND
      |                     ; Q2: 3(S)
      |                     ; Q3: 1(S1), 4(S2)
      |                     ; R1: 2(n)
      |                     ; R18: 2
      |                     ; R21: 2
      |                     ; R24: 2
      |                     ; R35: 2
      |                     ; R42: 2
      |                     ; R44: 2
      |                     ; R48: 2
      |                     ; U1: 8(CH7), 9(DGND), 14(AGND)
      |                     ; U2: 2(GND), 3(REF2), 4(RESERVED_GND)
      |                     ; U3: 2(GND), 3(REF2), 4(RESERVED_GND)
      |                     ; U4: 3(GND)
      |                     ; U5: 3(GND)
      |                     ; U6: 3(GND)
      |                     ; U7: 3(GND), 8(GND), 13(GND), 18(GND), 23(GND), 28(GND), 33(AGND), 38(GND)
      |                     ; U9: 4(VEE)
      |                     ; U10: 1(GNDP), 2(GNDP), 5(GNDP), 8(GNDP), 9(GNDP), 10(GNDP), 11(GNDP), 12(GNDP), 13(GNDP), 14(GNDP), 15(GNDP), 16(GNDP), 17(GNDP), 18(GNDP)
      |                     ; U11: 2(GND)
      |                     ; U12: 2(GND)
      | 接続部品数　　　　　; 72部品（部品番号で集計。同一ネット全体）
      | 接続端子数　　　　　; 99端子（423端子の部品対応表で集計。ラベル・境界ポートの重複は含めない）
      | この場所の端子数　　; 1端子／1部品（同名ラベルによる接続を除く）
      | 同階層同名ラベル数　; 75個（このラベル自身を含む）
      | 全階層の接続ラベル　; 87個（実際に同じノードへつながるラベル。名前が違う別名も含む）
      | 接続ルール　　　　　; 同じ階層の同じラベル名を仮想配線として結ぶ。別のSubsystem内とは名前だけでつながらず、明示的なConnection Portと配線をたどる。色は用途の表示であり接続を決めない。
      | 確認の範囲　　　　　; 現在の保存回路の端子・配線から求めた静的接続。抵抗やICの内部を導線として短絡せずに集計した。説明の更新は動作シミュレーション、タイミング、実部品の性能・実機動作を保証するものではない。
      | 記録の基準　　　　　; measurement_label_layout_20261022_r01/after_layout_graph.json。部品対応表は端子名の対応付けにのみ使用。
      | 
      | 【この説明欄の略語・記号】
      | 用語1　　　　　　　 ; DC：Direct Current（直流）。ここでは直流電源または直流成分。DCバイアスはコンデンサに重なる直流電圧を指す。
      | 用語2　　　　　　　 ; DC/DC：DC-to-DC Converter（直流電圧変換器）。直流入力を別の直流電圧へ変換する電源回路。絶縁の有無は個々の部品説明で確認する。
      | 用語3　　　　　　　 ; ADC：Analog-to-Digital Converter（アナログ・デジタル変換器）。測定電圧をデジタル値へ変換する回路。電流や温度も、センサーで電圧へ変換した後に読み取る。
      | 用語4　　　　　　　 ; IC：Integrated Circuit（集積回路）。複数の電子素子と機能を小さな半導体チップに集積した部品。
      | 用語5　　　　　　　 ; CH：Channel（測定チャネル）。CH0〜CH7はADCの入力番号であり、同時測定を意味しない。
      | 用語6　　　　　　　 ; MOSFET：Metal-Oxide-Semiconductor Field-Effect Transistor（金属・酸化膜・半導体構造の電界効果トランジスタ）。ゲートとソースの電圧でドレインとソースの導通を制御する素子。N-MOSはNチャネル型を表す。
      | 用語7　　　　　　　 ; LiFePO4：Lithium Iron Phosphate（リン酸鉄リチウム）。電池の正極材料を示す化学式。英語の頭文字を並べた略語ではない。
      | 用語8　　　　　　　 ; GND：Ground（回路の基準電位・電流帰路）。この図の共通基準。保護接地や大地への接続を意味するとは限らない。
      | 用語9　　　　　　　 ; AGND：Analog Ground（アナログ回路の基準端子）。アナログ部分の電流帰路。現図では共通GNDへ接続されるが、実装時の電流経路への配慮は別途必要。
      | 用語10　　　　　　　; DGND：Digital Ground（デジタル回路の基準端子）。デジタル部分の電流帰路。現図では共通GNDへ接続される。
      | 用語11　　　　　　　; VREF/REF：基準電圧を表す端子名。REFはReference（基準）の意味。ADCの変換尺度や電流アンプの出力基準に使う。REF1/REF2の接続電位は個別に確認する。
      | 用語12　　　　　　　; VCC/VDD/VEE/VS：ICの電源端子名。文字の歴史的な由来を現在の接続機能へ当てはめない。現回路のVEEはU8/U10では浮動基準SW、U9ではGND。各電圧・基準は端子と接続を参照する。
      | 用語13　　　　　　　; GNDP：U10の一次側電源の基準端子。絶縁電源の入力側GND。二次側基準VEE=SWと直接同一の導体ではない。
      | 用語14　　　　　　　; SW：Switching Node（スイッチング点）。主電力段の上下MOSFETとL1がつながる、電圧が高速に切り替わる点。GNDとは別電位。
  GND_Label_087 : ConnectionLabel  Description=|  Label=GND
      | この回路での名前　　; GND
      | 種別　　　　　　　　; ConnectionLabel
      | この回路での役割　　; 電池BT1の負極、太陽電池列の負極、制御・測定・保護回路のGNDを結ぶ共通の帰路。高側駆動の浮動帰路SWとは別のノード。
      | 共通帰路の代表接続　; BT1（充電先の蓄電池／51.2V 100Ah LiFePO4）: -
      |                     ; PV1（直列太陽電池列の負極側パネル／400W panel 1/2）: -
      |                     ; U7（RP2040搭載Pico W／SC0918）: 3(GND), 8(GND), 13(GND), 18(GND), 23(GND), 28(GND), 33(AGND), 38(GND)
      |                     ; U1（外付けADC／MCP3208-CI/SL）: 8(CH7), 9(DGND), 14(AGND)
      |                     ; P_U1（保護MOSFETを制御する保護IC／LTC4364IMS-1#PBF）: GND
      |                     ; Q2（同期整流降圧回路の下側スイッチ／TK9R6E15Q5,S1X）: 3(S)
      |                     ; U9（低側の光ゲートドライバ／ACPL-P346-560E）: 4(VEE)
      |                     ; U10（高側ゲート用の浮動電源を作る絶縁DC/DC／UCC14131QDWNRQ1）: 1(GNDP), 2(GNDP), 5(GNDP), 8(GNDP), 9(GNDP), 10(GNDP), 11(GNDP), 12(GNDP), 13(GNDP), 14(GNDP), 15(GNDP), 16(GNDP), 17(GNDP), 18(GNDP)
      | この場所の直接接続　; U3（L1直後の出力電流の検出アンプ／INA241A3IDDFR）: 4(RESERVED_GND)
      | 直接接続の範囲　　　; このラベルから実際の線・分岐・明示的な境界端子だけを追った接続。同名ラベルによる離れた場所への接続はこの欄に含めない。
      | 同一ネット全端子　　; BT1: -
      |                     ; C1: 2(n)
      |                     ; C2: 2(n)
      |                     ; C3: 2(n)
      |                     ; C4: 2(n)
      |                     ; C7: 2(n)
      |                     ; C8: 2(n)
      |                     ; C9: 2(n)
      |                     ; C10: 2(n)
      |                     ; C13: 2(n)
      |                     ; C14: 2(n)
      |                     ; C15: 2(n)
      |                     ; C16: 2(n)
      |                     ; C17: 2
      |                     ; C18: 2
      |                     ; C19: 2
      |                     ; C20: 2
      |                     ; C21: 2
      |                     ; C22: 2
      |                     ; C23: 2
      |                     ; C24: 2
      |                     ; C25: 2
      |                     ; C26: 2
      |                     ; C27: 2
      |                     ; C28: 2
      |                     ; C29: 2
      |                     ; C30: 2
      |                     ; C31: 2
      |                     ; C33: 2
      |                     ; C34: 2
      |                     ; C35: 2
      |                     ; C36: 2
      |                     ; C40: 2
      |                     ; C41: 2
      |                     ; C42: 2
      |                     ; C43: 2
      |                     ; C44: 2
      |                     ; C45: 2
      |                     ; C46: 2
      |                     ; C47: 2
      |                     ; C48: 2
      |                     ; D2: 2(A)
      |                     ; PV1: -
      |                     ; P_CHG: N
      |                     ; P_COUT: N
      |                     ; P_CTMR: N
      |                     ; P_D1: A
      |                     ; P_R3: 2
      |                     ; P_R8: 2
      |                     ; P_RSHDN_PD: 2
      |                     ; P_U1: GND
      |                     ; Q2: 3(S)
      |                     ; Q3: 1(S1), 4(S2)
      |                     ; R1: 2(n)
      |                     ; R18: 2
      |                     ; R21: 2
      |                     ; R24: 2
      |                     ; R35: 2
      |                     ; R42: 2
      |                     ; R44: 2
      |                     ; R48: 2
      |                     ; U1: 8(CH7), 9(DGND), 14(AGND)
      |                     ; U2: 2(GND), 3(REF2), 4(RESERVED_GND)
      |                     ; U3: 2(GND), 3(REF2), 4(RESERVED_GND)
      |                     ; U4: 3(GND)
      |                     ; U5: 3(GND)
      |                     ; U6: 3(GND)
      |                     ; U7: 3(GND), 8(GND), 13(GND), 18(GND), 23(GND), 28(GND), 33(AGND), 38(GND)
      |                     ; U9: 4(VEE)
      |                     ; U10: 1(GNDP), 2(GNDP), 5(GNDP), 8(GNDP), 9(GNDP), 10(GNDP), 11(GNDP), 12(GNDP), 13(GNDP), 14(GNDP), 15(GNDP), 16(GNDP), 17(GNDP), 18(GNDP)
      |                     ; U11: 2(GND)
      |                     ; U12: 2(GND)
      | 接続部品数　　　　　; 72部品（部品番号で集計。同一ネット全体）
      | 接続端子数　　　　　; 99端子（423端子の部品対応表で集計。ラベル・境界ポートの重複は含めない）
      | この場所の端子数　　; 1端子／1部品（同名ラベルによる接続を除く）
      | 同階層同名ラベル数　; 75個（このラベル自身を含む）
      | 全階層の接続ラベル　; 87個（実際に同じノードへつながるラベル。名前が違う別名も含む）
      | 接続ルール　　　　　; 同じ階層の同じラベル名を仮想配線として結ぶ。別のSubsystem内とは名前だけでつながらず、明示的なConnection Portと配線をたどる。色は用途の表示であり接続を決めない。
      | 確認の範囲　　　　　; 現在の保存回路の端子・配線から求めた静的接続。抵抗やICの内部を導線として短絡せずに集計した。説明の更新は動作シミュレーション、タイミング、実部品の性能・実機動作を保証するものではない。
      | 記録の基準　　　　　; measurement_label_layout_20261022_r01/after_layout_graph.json。部品対応表は端子名の対応付けにのみ使用。
      | 
      | 【この説明欄の略語・記号】
      | 用語1　　　　　　　 ; DC：Direct Current（直流）。ここでは直流電源または直流成分。DCバイアスはコンデンサに重なる直流電圧を指す。
      | 用語2　　　　　　　 ; DC/DC：DC-to-DC Converter（直流電圧変換器）。直流入力を別の直流電圧へ変換する電源回路。絶縁の有無は個々の部品説明で確認する。
      | 用語3　　　　　　　 ; ADC：Analog-to-Digital Converter（アナログ・デジタル変換器）。測定電圧をデジタル値へ変換する回路。電流や温度も、センサーで電圧へ変換した後に読み取る。
      | 用語4　　　　　　　 ; IC：Integrated Circuit（集積回路）。複数の電子素子と機能を小さな半導体チップに集積した部品。
      | 用語5　　　　　　　 ; CH：Channel（測定チャネル）。CH0〜CH7はADCの入力番号であり、同時測定を意味しない。
      | 用語6　　　　　　　 ; MOSFET：Metal-Oxide-Semiconductor Field-Effect Transistor（金属・酸化膜・半導体構造の電界効果トランジスタ）。ゲートとソースの電圧でドレインとソースの導通を制御する素子。N-MOSはNチャネル型を表す。
      | 用語7　　　　　　　 ; LiFePO4：Lithium Iron Phosphate（リン酸鉄リチウム）。電池の正極材料を示す化学式。英語の頭文字を並べた略語ではない。
      | 用語8　　　　　　　 ; GND：Ground（回路の基準電位・電流帰路）。この図の共通基準。保護接地や大地への接続を意味するとは限らない。
      | 用語9　　　　　　　 ; AGND：Analog Ground（アナログ回路の基準端子）。アナログ部分の電流帰路。現図では共通GNDへ接続されるが、実装時の電流経路への配慮は別途必要。
      | 用語10　　　　　　　; DGND：Digital Ground（デジタル回路の基準端子）。デジタル部分の電流帰路。現図では共通GNDへ接続される。
      | 用語11　　　　　　　; VREF/REF：基準電圧を表す端子名。REFはReference（基準）の意味。ADCの変換尺度や電流アンプの出力基準に使う。REF1/REF2の接続電位は個別に確認する。
      | 用語12　　　　　　　; VCC/VDD/VEE/VS：ICの電源端子名。文字の歴史的な由来を現在の接続機能へ当てはめない。現回路のVEEはU8/U10では浮動基準SW、U9ではGND。各電圧・基準は端子と接続を参照する。
      | 用語13　　　　　　　; GNDP：U10の一次側電源の基準端子。絶縁電源の入力側GND。二次側基準VEE=SWと直接同一の導体ではない。
      | 用語14　　　　　　　; SW：Switching Node（スイッチング点）。主電力段の上下MOSFETとL1がつながる、電圧が高速に切り替わる点。GNDとは別電位。
  GND_Label_088 : ConnectionLabel  Description=|  Label=GND
      | この回路での名前　　; GND
      | 種別　　　　　　　　; ConnectionLabel
      | この回路での役割　　; 電池BT1の負極、太陽電池列の負極、制御・測定・保護回路のGNDを結ぶ共通の帰路。高側駆動の浮動帰路SWとは別のノード。
      | 共通帰路の代表接続　; BT1（充電先の蓄電池／51.2V 100Ah LiFePO4）: -
      |                     ; PV1（直列太陽電池列の負極側パネル／400W panel 1/2）: -
      |                     ; U7（RP2040搭載Pico W／SC0918）: 3(GND), 8(GND), 13(GND), 18(GND), 23(GND), 28(GND), 33(AGND), 38(GND)
      |                     ; U1（外付けADC／MCP3208-CI/SL）: 8(CH7), 9(DGND), 14(AGND)
      |                     ; P_U1（保護MOSFETを制御する保護IC／LTC4364IMS-1#PBF）: GND
      |                     ; Q2（同期整流降圧回路の下側スイッチ／TK9R6E15Q5,S1X）: 3(S)
      |                     ; U9（低側の光ゲートドライバ／ACPL-P346-560E）: 4(VEE)
      |                     ; U10（高側ゲート用の浮動電源を作る絶縁DC/DC／UCC14131QDWNRQ1）: 1(GNDP), 2(GNDP), 5(GNDP), 8(GNDP), 9(GNDP), 10(GNDP), 11(GNDP), 12(GNDP), 13(GNDP), 14(GNDP), 15(GNDP), 16(GNDP), 17(GNDP), 18(GNDP)
      | この場所の直接接続　; U4（電池温度センサー／TMP235A2DBZR）: 3(GND)
      | 直接接続の範囲　　　; このラベルから実際の線・分岐・明示的な境界端子だけを追った接続。同名ラベルによる離れた場所への接続はこの欄に含めない。
      | 同一ネット全端子　　; BT1: -
      |                     ; C1: 2(n)
      |                     ; C2: 2(n)
      |                     ; C3: 2(n)
      |                     ; C4: 2(n)
      |                     ; C7: 2(n)
      |                     ; C8: 2(n)
      |                     ; C9: 2(n)
      |                     ; C10: 2(n)
      |                     ; C13: 2(n)
      |                     ; C14: 2(n)
      |                     ; C15: 2(n)
      |                     ; C16: 2(n)
      |                     ; C17: 2
      |                     ; C18: 2
      |                     ; C19: 2
      |                     ; C20: 2
      |                     ; C21: 2
      |                     ; C22: 2
      |                     ; C23: 2
      |                     ; C24: 2
      |                     ; C25: 2
      |                     ; C26: 2
      |                     ; C27: 2
      |                     ; C28: 2
      |                     ; C29: 2
      |                     ; C30: 2
      |                     ; C31: 2
      |                     ; C33: 2
      |                     ; C34: 2
      |                     ; C35: 2
      |                     ; C36: 2
      |                     ; C40: 2
      |                     ; C41: 2
      |                     ; C42: 2
      |                     ; C43: 2
      |                     ; C44: 2
      |                     ; C45: 2
      |                     ; C46: 2
      |                     ; C47: 2
      |                     ; C48: 2
      |                     ; D2: 2(A)
      |                     ; PV1: -
      |                     ; P_CHG: N
      |                     ; P_COUT: N
      |                     ; P_CTMR: N
      |                     ; P_D1: A
      |                     ; P_R3: 2
      |                     ; P_R8: 2
      |                     ; P_RSHDN_PD: 2
      |                     ; P_U1: GND
      |                     ; Q2: 3(S)
      |                     ; Q3: 1(S1), 4(S2)
      |                     ; R1: 2(n)
      |                     ; R18: 2
      |                     ; R21: 2
      |                     ; R24: 2
      |                     ; R35: 2
      |                     ; R42: 2
      |                     ; R44: 2
      |                     ; R48: 2
      |                     ; U1: 8(CH7), 9(DGND), 14(AGND)
      |                     ; U2: 2(GND), 3(REF2), 4(RESERVED_GND)
      |                     ; U3: 2(GND), 3(REF2), 4(RESERVED_GND)
      |                     ; U4: 3(GND)
      |                     ; U5: 3(GND)
      |                     ; U6: 3(GND)
      |                     ; U7: 3(GND), 8(GND), 13(GND), 18(GND), 23(GND), 28(GND), 33(AGND), 38(GND)
      |                     ; U9: 4(VEE)
      |                     ; U10: 1(GNDP), 2(GNDP), 5(GNDP), 8(GNDP), 9(GNDP), 10(GNDP), 11(GNDP), 12(GNDP), 13(GNDP), 14(GNDP), 15(GNDP), 16(GNDP), 17(GNDP), 18(GNDP)
      |                     ; U11: 2(GND)
      |                     ; U12: 2(GND)
      | 接続部品数　　　　　; 72部品（部品番号で集計。同一ネット全体）
      | 接続端子数　　　　　; 99端子（423端子の部品対応表で集計。ラベル・境界ポートの重複は含めない）
      | この場所の端子数　　; 1端子／1部品（同名ラベルによる接続を除く）
      | 同階層同名ラベル数　; 75個（このラベル自身を含む）
      | 全階層の接続ラベル　; 87個（実際に同じノードへつながるラベル。名前が違う別名も含む）
      | 接続ルール　　　　　; 同じ階層の同じラベル名を仮想配線として結ぶ。別のSubsystem内とは名前だけでつながらず、明示的なConnection Portと配線をたどる。色は用途の表示であり接続を決めない。
